simulink model "s_c107m32k_vlbi"  (R2018a)
(part 4 of 201)

      mask help: A 32-bit software-accessible register. Can be divided into bitfields of varying widths and types using the fields in the block mask.
      mask init:
      | swreg_init(gcb)
      settings: AttributesFormatString=2 inputs:uf16.0,uf16.0 = 32 bits
      mask TypeOptions io_dir: To Processor | From Processor
      mask Callback io_dir:
      | mask_enables = get_param(gcb, 'MaskEnables');
      | mask_names = get_param(gcb, 'MaskNames');
      | if strcmp(get_param(gcb, 'io_dir'), 'To Processor'),
      |     mask_enables{ismember(mask_names, 'sample_period')} = 'off';
      | else
      |     mask_enables{ismember(mask_names, 'sample_period')} = 'on';
      | end
      | set_param(gcb, 'MaskEnables', mask_enables);
      mask DialogControl ParameterTabVar0 Prompt: Setup
  tx_metadata : Subsystem  Tag=xps:sw_reg  AncestorBlock=xps_library/Memory/software_register  mask(swreg){io_dir=From Processor, io_delay=0, init_val=0, sample_period=1, names=[porttx board_id], bitwidths=[16 8], bin_pts=0, arith_types=0, sim_port=off, show_format=on}
      mask prompts: io_dir "I/O direction"; io_delay "I/O delay"; init_val "Initial Value"; sample_period "Sample period"; names "Bitfield names [msb...lsb]"; bitwidths "Bitfield widths"; bin_pts "Bitfield binary pts"; arith_types "Bitfield types, ufix=0, fix=1, bool=2"; sim_port "Provide sim input/output?"; show_format "Print format string?"
      mask help: A 32-bit software-accessible register. Can be divided into bitfields of varying widths and types using the fields in the block mask.
      mask init:
      | swreg_init(gcb)
      settings: AttributesFormatString=2 inputs:uf16.0,uf8.0 = 24 bits
      mask TypeOptions io_dir: To Processor | From Processor
      mask Callback io_dir:
      | mask_enables = get_param(gcb, 'MaskEnables');
      | mask_names = get_param(gcb, 'MaskNames');
      | if strcmp(get_param(gcb, 'io_dir'), 'To Processor'),
      |     mask_enables{ismember(mask_names, 'sample_period')} = 'off';
      | else
      |     mask_enables{ismember(mask_names, 'sample_period')} = 'on';
      | end
      | set_param(gcb, 'MaskEnables', mask_enables);
      mask DialogControl ParameterTabVar0 Prompt: Setup
  unpack : Subsystem
  unpack_status : Subsystem  Tag=xps:sw_reg  AncestorBlock=xps_library/Memory/software_register  mask(swreg){io_dir=To Processor, io_delay=0, init_val=0, sample_period=1, names=[magic_err_cnt header_err_cnt pad_err_cnt pkt_len_err_cnt time_err_cnt], bitwidths=6, bin_pts=0, arith_types=0, sim_port=off, show_format=on}
      mask prompts: io_dir "I/O direction"; io_delay "I/O delay"; init_val "Initial Value"; sample_period "Sample period"; names "Bitfield names [msb...lsb]"; bitwidths "Bitfield widths"; bin_pts "Bitfield binary pts"; arith_types "Bitfield types, ufix=0, fix=1, bool=2"; sim_port "Provide sim input/output?"; show_format "Print format string?"
      mask help: A 32-bit software-accessible register. Can be divided into bitfields of varying widths and types using the fields in the block mask.
      mask init:
      | swreg_init(gcb)
      settings: AttributesFormatString=5 outputs:uf6.0,uf6.0,uf6.0,uf6.0,uf6.0 = 30 bits
      mask TypeOptions io_dir: To Processor | From Processor
      mask Callback io_dir:
      | mask_enables = get_param(gcb, 'MaskEnables');
      | mask_names = get_param(gcb, 'MaskNames');
      | if strcmp(get_param(gcb, 'io_dir'), 'To Processor'),
      |     mask_enables{ismember(mask_names, 'sample_period')} = 'off';
      | else
      |     mask_enables{ismember(mask_names, 'sample_period')} = 'on';
      | end
      | set_param(gcb, 'MaskEnables', mask_enables);
      mask DialogControl ParameterTabVar0 Prompt: Setup
  unpack_status1 : Subsystem  Tag=xps:sw_reg  AncestorBlock=xps_library/Memory/software_register  mask(swreg){io_dir=To Processor, io_delay=0, init_val=0, sample_period=1, names=pkt_cnt, bitwidths=32, bin_pts=0, arith_types=0, sim_port=off, show_format=on}
      mask prompts: io_dir "I/O direction"; io_delay "I/O delay"; init_val "Initial Value"; sample_period "Sample period"; names "Bitfield names [msb...lsb]"; bitwidths "Bitfield widths"; bin_pts "Bitfield binary pts"; arith_types "Bitfield types, ufix=0, fix=1, bool=2"; sim_port "Provide sim input/output?"; show_format "Print format string?"
      mask help: A 32-bit software-accessible register. Can be divided into bitfields of varying widths and types using the fields in the block mask.
      mask init:
      | swreg_init(gcb)
      settings: AttributesFormatString=1output:uf32.0 = 32 bits
      mask TypeOptions io_dir: To Processor | From Processor
      mask Callback io_dir:
      | mask_enables = get_param(gcb, 'MaskEnables');
      | mask_names = get_param(gcb, 'MaskNames');
      | if strcmp(get_param(gcb, 'io_dir'), 'To Processor'),
      |     mask_enables{ismember(mask_names, 'sample_period')} = 'off';
      | else
      |     mask_enables{ismember(mask_names, 'sample_period')} = 'on';
      | end
      | set_param(gcb, 'MaskEnables', mask_enables);
      mask DialogControl ParameterTabVar0 Prompt: Setup
  we_delay1 : Subsystem  Tag=cmac_delinked  Commented=on  mask(pipeline){csp_latency=2}
      mask prompts: csp_latency "Latency"
      mask help:
      | An explicitly laid-out delay line to avoid mapping to SRL16s
      | for use in pipelining to help achieve timing closure.
      mask init:
      | pipeline_init(gcb,'latency',csp_latency);
      settings: AttributesFormatString=Latency = %<latency>
      mask Display:
      | port_label('input', 1, 'd');
      | port_label('output', 1, 'q');
      | disp(['Z^-', num2str(csp_latency)]);
  we_delay10 : Subsystem  Tag=cmac_delinked  Commented=on  mask(pipeline){csp_latency=1}
      mask prompts: csp_latency "Latency"
      mask help:
      | An explicitly laid-out delay line to avoid mapping to SRL16s
      | for use in pipelining to help achieve timing closure.
      mask init:
      | pipeline_init(gcb,'latency',csp_latency);
      settings: AttributesFormatString=Latency = %<latency>
      mask Display:
      | port_label('input', 1, 'd');
      | port_label('output', 1, 'q');
      | disp(['Z^-', num2str(csp_latency)]);
  we_delay11 : Subsystem  Tag=cmac_delinked  Commented=on  mask(pipeline){csp_latency=1}
      mask prompts: csp_latency "Latency"
      mask help:
      | An explicitly laid-out delay line to avoid mapping to SRL16s
      | for use in pipelining to help achieve timing closure.
      mask init:
      | pipeline_init(gcb,'latency',csp_latency);
      settings: AttributesFormatString=Latency = %<latency>
      mask Display:
      | port_label('input', 1, 'd');
      | port_label('output', 1, 'q');
      | disp(['Z^-', num2str(csp_latency)]);
  we_delay112 : Subsystem  Tag=cmac_delinked  mask(pipeline){csp_latency=2}
      mask prompts: csp_latency "Latency"
      mask help:
      | An explicitly laid-out delay line to avoid mapping to SRL16s
      | for use in pipelining to help achieve timing closure.
      mask init:
      | pipeline_init(gcb,'latency',csp_latency);
      settings: AttributesFormatString=Latency = %<latency>
      mask Display:
      | port_label('input', 1, 'd');
      | port_label('output', 1, 'q');
      | disp(['Z^-', num2str(csp_latency)]);
  we_delay113 : Subsystem  Tag=cmac_delinked  mask(pipeline){csp_latency=2}
      mask prompts: csp_latency "Latency"
      mask help:
      | An explicitly laid-out delay line to avoid mapping to SRL16s
      | for use in pipelining to help achieve timing closure.
      mask init:
      | pipeline_init(gcb,'latency',csp_latency);
      settings: AttributesFormatString=Latency = %<latency>
      mask Display:
      | port_label('input', 1, 'd');
      | port_label('output', 1, 'q');
      | disp(['Z^-', num2str(csp_latency)]);
  we_delay114 : Subsystem  Tag=cmac_delinked  mask(pipeline){csp_latency=2}
      mask prompts: csp_latency "Latency"
      mask help:
      | An explicitly laid-out delay line to avoid mapping to SRL16s
      | for use in pipelining to help achieve timing closure.
      mask init:
      | pipeline_init(gcb,'latency',csp_latency);
      settings: AttributesFormatString=Latency = %<latency>
      mask Display:
      | port_label('input', 1, 'd');
      | port_label('output', 1, 'q');
      | disp(['Z^-', num2str(csp_latency)]);
  we_delay115 : Subsystem  Tag=cmac_delinked  mask(pipeline){csp_latency=2}
      mask prompts: csp_latency "Latency"
      mask help:
      | An explicitly laid-out delay line to avoid mapping to SRL16s
      | for use in pipelining to help achieve timing closure.
      mask init:
      | pipeline_init(gcb,'latency',csp_latency);
      settings: AttributesFormatString=Latency = %<latency>
      mask Display:
      | port_label('input', 1, 'd');
      | port_label('output', 1, 'q');
      | disp(['Z^-', num2str(csp_latency)]);
  we_delay116 : Subsystem  Tag=cmac_delinked  mask(pipeline){csp_latency=2}
      mask prompts: csp_latency "Latency"
      mask help:
      | An explicitly laid-out delay line to avoid mapping to SRL16s
      | for use in pipelining to help achieve timing closure.
      mask init:
      | pipeline_init(gcb,'latency',csp_latency);
      settings: AttributesFormatString=Latency = %<latency>
      mask Display:
      | port_label('input', 1, 'd');
      | port_label('output', 1, 'q');
      | disp(['Z^-', num2str(csp_latency)]);
  we_delay117 : Subsystem  Tag=cmac_delinked  mask(pipeline){csp_latency=2}
      mask prompts: csp_latency "Latency"
      mask help:
      | An explicitly laid-out delay line to avoid mapping to SRL16s
      | for use in pipelining to help achieve timing closure.
      mask init:
      | pipeline_init(gcb,'latency',csp_latency);
      settings: AttributesFormatString=Latency = %<latency>
      mask Display:
      | port_label('input', 1, 'd');
      | port_label('output', 1, 'q');
      | disp(['Z^-', num2str(csp_latency)]);
  we_delay12 : Subsystem  Tag=cmac_delinked  Commented=on  mask(pipeline){csp_latency=1}
      mask prompts: csp_latency "Latency"
      mask help:
      | An explicitly laid-out delay line to avoid mapping to SRL16s
      | for use in pipelining to help achieve timing closure.
      mask init:
      | pipeline_init(gcb,'latency',csp_latency);
      settings: AttributesFormatString=Latency = %<latency>
      mask Display:
      | port_label('input', 1, 'd');
      | port_label('output', 1, 'q');
      | disp(['Z^-', num2str(csp_latency)]);
  we_delay124 : Subsystem  Tag=cmac_delinked  mask(pipeline){csp_latency=2}
      mask prompts: csp_latency "Latency"
      mask help:
      | An explicitly laid-out delay line to avoid mapping to SRL16s
      | for use in pipelining to help achieve timing closure.
      mask init:
      | pipeline_init(gcb,'latency',csp_latency);
      settings: AttributesFormatString=Latency = %<latency>
      mask Display:
      | port_label('input', 1, 'd');
      | port_label('output', 1, 'q');
      | disp(['Z^-', num2str(csp_latency)]);
  we_delay126 : Subsystem  Tag=cmac_delinked  mask(pipeline){csp_latency=2}
      mask prompts: csp_latency "Latency"
      mask help:
      | An explicitly laid-out delay line to avoid mapping to SRL16s
      | for use in pipelining to help achieve timing closure.
      mask init:
      | pipeline_init(gcb,'latency',csp_latency);
      settings: AttributesFormatString=Latency = %<latency>
      mask Display:
      | port_label('input', 1, 'd');
      | port_label('output', 1, 'q');
      | disp(['Z^-', num2str(csp_latency)]);
  we_delay13 : Subsystem  Tag=cmac_delinked  mask(pipeline){csp_latency=2}
      mask prompts: csp_latency "Latency"
      mask help:
      | An explicitly laid-out delay line to avoid mapping to SRL16s
      | for use in pipelining to help achieve timing closure.
      mask init:
      | pipeline_init(gcb,'latency',csp_latency);
      settings: AttributesFormatString=Latency = %<latency>
      mask Display:
      | port_label('input', 1, 'd');
      | port_label('output', 1, 'q');
      | disp(['Z^-', num2str(csp_latency)]);
  we_delay14 : Subsystem  Tag=cmac_delinked  Commented=on  mask(pipeline){csp_latency=1}
      mask prompts: csp_latency "Latency"
      mask help:
      | An explicitly laid-out delay line to avoid mapping to SRL16s
      | for use in pipelining to help achieve timing closure.
      mask init:
      | pipeline_init(gcb,'latency',csp_latency);
      settings: AttributesFormatString=Latency = %<latency>
      mask Display:
      | port_label('input', 1, 'd');
      | port_label('output', 1, 'q');
      | disp(['Z^-', num2str(csp_latency)]);
  we_delay15 : Subsystem  Tag=cmac_delinked  Commented=on  mask(pipeline){csp_latency=1}
      mask prompts: csp_latency "Latency"
      mask help:
      | An explicitly laid-out delay line to avoid mapping to SRL16s
      | for use in pipelining to help achieve timing closure.
      mask init:
      | pipeline_init(gcb,'latency',csp_latency);
      settings: AttributesFormatString=Latency = %<latency>
      mask Display:
      | port_label('input', 1, 'd');
      | port_label('output', 1, 'q');
      | disp(['Z^-', num2str(csp_latency)]);
  we_delay2 : Subsystem  Tag=cmac_delinked  Commented=on  mask(pipeline){csp_latency=1}
      mask prompts: csp_latency "Latency"
      mask help:
      | An explicitly laid-out delay line to avoid mapping to SRL16s
      | for use in pipelining to help achieve timing closure.
      mask init:
      | pipeline_init(gcb,'latency',csp_latency);
      settings: AttributesFormatString=Latency = %<latency>
      mask Display:
      | port_label('input', 1, 'd');
      | port_label('output', 1, 'q');
      | disp(['Z^-', num2str(csp_latency)]);
  we_delay25 : Subsystem  Tag=cmac_delinked  Commented=on  mask(pipeline){csp_latency=2}
      mask prompts: csp_latency "Latency"
      mask help:
      | An explicitly laid-out delay line to avoid mapping to SRL16s
      | for use in pipelining to help achieve timing closure.
      mask init:
      | pipeline_init(gcb,'latency',csp_latency);
      settings: AttributesFormatString=Latency = %<latency>
      mask Display:
      | port_label('input', 1, 'd');
      | port_label('output', 1, 'q');
      | disp(['Z^-', num2str(csp_latency)]);
  we_delay3 : Subsystem  Tag=cmac_delinked  Commented=on  mask(pipeline){csp_latency=1}
      mask prompts: csp_latency "Latency"
      mask help:
      | An explicitly laid-out delay line to avoid mapping to SRL16s
      | for use in pipelining to help achieve timing closure.
      mask init:
      | pipeline_init(gcb,'latency',csp_latency);
      settings: AttributesFormatString=Latency = %<latency>
      mask Display:
      | port_label('input', 1, 'd');
      | port_label('output', 1, 'q');
      | disp(['Z^-', num2str(csp_latency)]);
  we_delay35 : Subsystem  Tag=cmac_delinked  Commented=on  mask(pipeline){csp_latency=2}
      mask prompts: csp_latency "Latency"
      mask help:
      | An explicitly laid-out delay line to avoid mapping to SRL16s
      | for use in pipelining to help achieve timing closure.
      mask init:
      | pipeline_init(gcb,'latency',csp_latency);
      settings: AttributesFormatString=Latency = %<latency>
      mask Display:
      | port_label('input', 1, 'd');
      | port_label('output', 1, 'q');
      | disp(['Z^-', num2str(csp_latency)]);
  we_delay37 : Subsystem  Tag=cmac_delinked  mask(pipeline){csp_latency=2}
      mask prompts: csp_latency "Latency"
      mask help:
      | An explicitly laid-out delay line to avoid mapping to SRL16s
      | for use in pipelining to help achieve timing closure.
      mask init:
      | pipeline_init(gcb,'latency',csp_latency);
      settings: AttributesFormatString=Latency = %<latency>
      mask Display:
      | port_label('input', 1, 'd');
      | port_label('output', 1, 'q');
      | disp(['Z^-', num2str(csp_latency)]);
  we_delay38 : Subsystem  Tag=cmac_delinked  mask(pipeline){csp_latency=2}
      mask prompts: csp_latency "Latency"
      mask help:
      | An explicitly laid-out delay line to avoid mapping to SRL16s
      | for use in pipelining to help achieve timing closure.
      mask init:
      | pipeline_init(gcb,'latency',csp_latency);
      settings: AttributesFormatString=Latency = %<latency>
      mask Display:
      | port_label('input', 1, 'd');
      | port_label('output', 1, 'q');
      | disp(['Z^-', num2str(csp_latency)]);
  we_delay39 : Subsystem  Tag=cmac_delinked  mask(pipeline){csp_latency=2}
      mask prompts: csp_latency "Latency"
      mask help:
      | An explicitly laid-out delay line to avoid mapping to SRL16s
      | for use in pipelining to help achieve timing closure.
      mask init:
      | pipeline_init(gcb,'latency',csp_latency);
      settings: AttributesFormatString=Latency = %<latency>
      mask Display:
      | port_label('input', 1, 'd');
      | port_label('output', 1, 'q');
      | disp(['Z^-', num2str(csp_latency)]);
  we_delay4 : Subsystem  Tag=cmac_delinked  Commented=on  mask(pipeline){csp_latency=1}
      mask prompts: csp_latency "Latency"
      mask help:
      | An explicitly laid-out delay line to avoid mapping to SRL16s
      | for use in pipelining to help achieve timing closure.
      mask init:
      | pipeline_init(gcb,'latency',csp_latency);
      settings: AttributesFormatString=Latency = %<latency>
      mask Display:
      | port_label('input', 1, 'd');
      | port_label('output', 1, 'q');
      | disp(['Z^-', num2str(csp_latency)]);
  we_delay41 : Subsystem  Tag=cmac_delinked  mask(pipeline){csp_latency=2}
      mask prompts: csp_latency "Latency"
      mask help:
      | An explicitly laid-out delay line to avoid mapping to SRL16s
      | for use in pipelining to help achieve timing closure.
      mask init:
      | pipeline_init(gcb,'latency',csp_latency);
      settings: AttributesFormatString=Latency = %<latency>
      mask Display:
      | port_label('input', 1, 'd');
      | port_label('output', 1, 'q');
      | disp(['Z^-', num2str(csp_latency)]);
  we_delay47 : Subsystem  Tag=cmac_delinked  mask(pipeline){csp_latency=2}
      mask prompts: csp_latency "Latency"
      mask help:
      | An explicitly laid-out delay line to avoid mapping to SRL16s
      | for use in pipelining to help achieve timing closure.
      mask init:
      | pipeline_init(gcb,'latency',csp_latency);
      settings: AttributesFormatString=Latency = %<latency>
      mask Display:
      | port_label('input', 1, 'd');
      | port_label('output', 1, 'q');
      | disp(['Z^-', num2str(csp_latency)]);
  we_delay48 : Subsystem  Tag=cmac_delinked  mask(pipeline){csp_latency=2}
      mask prompts: csp_latency "Latency"
      mask help:
      | An explicitly laid-out delay line to avoid mapping to SRL16s
      | for use in pipelining to help achieve timing closure.
      mask init:
      | pipeline_init(gcb,'latency',csp_latency);
      settings: AttributesFormatString=Latency = %<latency>
      mask Display:
      | port_label('input', 1, 'd');
      | port_label('output', 1, 'q');
      | disp(['Z^-', num2str(csp_latency)]);
  we_delay49 : Subsystem  Tag=cmac_delinked  mask(pipeline){csp_latency=2}
      mask prompts: csp_latency "Latency"
      mask help:
      | An explicitly laid-out delay line to avoid mapping to SRL16s
      | for use in pipelining to help achieve timing closure.
      mask init:
      | pipeline_init(gcb,'latency',csp_latency);
      settings: AttributesFormatString=Latency = %<latency>
      mask Display:
      | port_label('input', 1, 'd');
      | port_label('output', 1, 'q');
      | disp(['Z^-', num2str(csp_latency)]);
  we_delay5 : Subsystem  Tag=cmac_delinked  Commented=on  mask(pipeline){csp_latency=1}
      mask prompts: csp_latency "Latency"
      mask help:
      | An explicitly laid-out delay line to avoid mapping to SRL16s
      | for use in pipelining to help achieve timing closure.
      mask init:
      | pipeline_init(gcb,'latency',csp_latency);
      settings: AttributesFormatString=Latency = %<latency>
      mask Display:
      | port_label('input', 1, 'd');
      | port_label('output', 1, 'q');
      | disp(['Z^-', num2str(csp_latency)]);
  we_delay50 : Subsystem  Tag=cmac_delinked  mask(pipeline){csp_latency=2}
      mask prompts: csp_latency "Latency"
      mask help:
      | An explicitly laid-out delay line to avoid mapping to SRL16s
      | for use in pipelining to help achieve timing closure.
      mask init:
      | pipeline_init(gcb,'latency',csp_latency);
      settings: AttributesFormatString=Latency = %<latency>
      mask Display:
      | port_label('input', 1, 'd');
      | port_label('output', 1, 'q');
      | disp(['Z^-', num2str(csp_latency)]);
  we_delay54 : Subsystem  Tag=cmac_delinked  Commented=on  mask(pipeline){csp_latency=2}
      mask prompts: csp_latency "Latency"
      mask help:
      | An explicitly laid-out delay line to avoid mapping to SRL16s
      | for use in pipelining to help achieve timing closure.
      mask init:
      | pipeline_init(gcb,'latency',csp_latency);
      settings: AttributesFormatString=Latency = %<latency>
      mask Display:
      | port_label('input', 1, 'd');
      | port_label('output', 1, 'q');
      | disp(['Z^-', num2str(csp_latency)]);
  we_delay55 : Subsystem  Tag=cmac_delinked  Commented=on  mask(pipeline){csp_latency=2}
      mask prompts: csp_latency "Latency"
      mask help:
      | An explicitly laid-out delay line to avoid mapping to SRL16s
      | for use in pipelining to help achieve timing closure.
      mask init:
      | pipeline_init(gcb,'latency',csp_latency);
      settings: AttributesFormatString=Latency = %<latency>
      mask Display:
      | port_label('input', 1, 'd');
      | port_label('output', 1, 'q');
      | disp(['Z^-', num2str(csp_latency)]);
  we_delay56 : Subsystem  Tag=cmac_delinked  Commented=on  mask(pipeline){csp_latency=2}
      mask prompts: csp_latency "Latency"
      mask help:
      | An explicitly laid-out delay line to avoid mapping to SRL16s
      | for use in pipelining to help achieve timing closure.
      mask init:
      | pipeline_init(gcb,'latency',csp_latency);
      settings: AttributesFormatString=Latency = %<latency>
      mask Display:
      | port_label('input', 1, 'd');
      | port_label('output', 1, 'q');
      | disp(['Z^-', num2str(csp_latency)]);
  we_delay57 : Subsystem  Tag=cmac_delinked  Commented=on  mask(pipeline){csp_latency=2}
      mask prompts: csp_latency "Latency"
      mask help:
      | An explicitly laid-out delay line to avoid mapping to SRL16s
      | for use in pipelining to help achieve timing closure.
      mask init:
      | pipeline_init(gcb,'latency',csp_latency);
      settings: AttributesFormatString=Latency = %<latency>
      mask Display:
      | port_label('input', 1, 'd');
      | port_label('output', 1, 'q');
      | disp(['Z^-', num2str(csp_latency)]);
  we_delay6 : Subsystem  Tag=cmac_delinked  Commented=on  mask(pipeline){csp_latency=1}
      mask prompts: csp_latency "Latency"
      mask help:
      | An explicitly laid-out delay line to avoid mapping to SRL16s
      | for use in pipelining to help achieve timing closure.
      mask init:
      | pipeline_init(gcb,'latency',csp_latency);
      settings: AttributesFormatString=Latency = %<latency>
      mask Display:
      | port_label('input', 1, 'd');
      | port_label('output', 1, 'q');
      | disp(['Z^-', num2str(csp_latency)]);
  we_delay68 : Subsystem  Tag=cmac_delinked  Commented=on  mask(pipeline){csp_latency=2}
      mask prompts: csp_latency "Latency"
      mask help:
      | An explicitly laid-out delay line to avoid mapping to SRL16s
      | for use in pipelining to help achieve timing closure.
      mask init:
      | pipeline_init(gcb,'latency',csp_latency);
      settings: AttributesFormatString=Latency = %<latency>
      mask Display:
      | port_label('input', 1, 'd');
      | port_label('output', 1, 'q');
      | disp(['Z^-', num2str(csp_latency)]);
  we_delay69 : Subsystem  Tag=cmac_delinked  Commented=on  mask(pipeline){csp_latency=2}
      mask prompts: csp_latency "Latency"
      mask help:
      | An explicitly laid-out delay line to avoid mapping to SRL16s
      | for use in pipelining to help achieve timing closure.
      mask init:
      | pipeline_init(gcb,'latency',csp_latency);
      settings: AttributesFormatString=Latency = %<latency>
      mask Display:
      | port_label('input', 1, 'd');
      | port_label('output', 1, 'q');
      | disp(['Z^-', num2str(csp_latency)]);
  we_delay7 : Subsystem  Tag=cmac_delinked  Commented=on  mask(pipeline){csp_latency=1}
      mask prompts: csp_latency "Latency"
      mask help:
      | An explicitly laid-out delay line to avoid mapping to SRL16s
      | for use in pipelining to help achieve timing closure.
      mask init:
      | pipeline_init(gcb,'latency',csp_latency);
      settings: AttributesFormatString=Latency = %<latency>
      mask Display:
      | port_label('input', 1, 'd');
      | port_label('output', 1, 'q');
      | disp(['Z^-', num2str(csp_latency)]);
  we_delay77 : Subsystem  Tag=cmac_delinked  mask(pipeline){csp_latency=2}
      mask prompts: csp_latency "Latency"
      mask help:
      | An explicitly laid-out delay line to avoid mapping to SRL16s
      | for use in pipelining to help achieve timing closure.
      mask init:
      | pipeline_init(gcb,'latency',csp_latency);
      settings: AttributesFormatString=Latency = %<latency>
      mask Display:
      | port_label('input', 1, 'd');
      | port_label('output', 1, 'q');
      | disp(['Z^-', num2str(csp_latency)]);
  we_delay78 : Subsystem  Tag=cmac_delinked  mask(pipeline){csp_latency=2}
      mask prompts: csp_latency "Latency"
      mask help:
      | An explicitly laid-out delay line to avoid mapping to SRL16s
      | for use in pipelining to help achieve timing closure.
      mask init:
      | pipeline_init(gcb,'latency',csp_latency);
      settings: AttributesFormatString=Latency = %<latency>
      mask Display:
      | port_label('input', 1, 'd');
      | port_label('output', 1, 'q');
      | disp(['Z^-', num2str(csp_latency)]);
  we_delay79 : Subsystem  Tag=cmac_delinked  Commented=on  mask(pipeline){csp_latency=2}
      mask prompts: csp_latency "Latency"
      mask help:
      | An explicitly laid-out delay line to avoid mapping to SRL16s
      | for use in pipelining to help achieve timing closure.
      mask init:
      | pipeline_init(gcb,'latency',csp_latency);
      settings: AttributesFormatString=Latency = %<latency>
      mask Display:
      | port_label('input', 1, 'd');
      | port_label('output', 1, 'q');
      | disp(['Z^-', num2str(csp_latency)]);
  we_delay8 : Subsystem  Tag=cmac_delinked  Commented=on  mask(pipeline){csp_latency=1}
      mask prompts: csp_latency "Latency"
      mask help:
      | An explicitly laid-out delay line to avoid mapping to SRL16s
      | for use in pipelining to help achieve timing closure.
      mask init:
      | pipeline_init(gcb,'latency',csp_latency);
      settings: AttributesFormatString=Latency = %<latency>
      mask Display:
      | port_label('input', 1, 'd');
      | port_label('output', 1, 'q');
      | disp(['Z^-', num2str(csp_latency)]);
  we_delay80 : Subsystem  Tag=cmac_delinked  Commented=on  mask(pipeline){csp_latency=2}
      mask prompts: csp_latency "Latency"
      mask help:
      | An explicitly laid-out delay line to avoid mapping to SRL16s
      | for use in pipelining to help achieve timing closure.
      mask init:
      | pipeline_init(gcb,'latency',csp_latency);
      settings: AttributesFormatString=Latency = %<latency>
      mask Display:
      | port_label('input', 1, 'd');
      | port_label('output', 1, 'q');
      | disp(['Z^-', num2str(csp_latency)]);
  we_delay81 : Subsystem  Tag=cmac_delinked  Commented=on  mask(pipeline){csp_latency=2}
      mask prompts: csp_latency "Latency"
      mask help:
      | An explicitly laid-out delay line to avoid mapping to SRL16s
      | for use in pipelining to help achieve timing closure.
      mask init:
      | pipeline_init(gcb,'latency',csp_latency);
      settings: AttributesFormatString=Latency = %<latency>
      mask Display:
      | port_label('input', 1, 'd');
      | port_label('output', 1, 'q');
      | disp(['Z^-', num2str(csp_latency)]);
  we_delay9 : Subsystem  Tag=cmac_delinked  Commented=on  mask(pipeline){csp_latency=1}
      mask prompts: csp_latency "Latency"
      mask help:
      | An explicitly laid-out delay line to avoid mapping to SRL16s
      | for use in pipelining to help achieve timing closure.
      mask init:
      | pipeline_init(gcb,'latency',csp_latency);
      settings: AttributesFormatString=Latency = %<latency>
      mask Display:
      | port_label('input', 1, 'd');
      | port_label('output', 1, 'q');
      | disp(['Z^-', num2str(csp_latency)]);
  x_setup : Subsystem  Tag=xps:sw_reg  AncestorBlock=xps_library/Memory/software_register  mask(swreg){io_dir=From Processor, io_delay=0, init_val=0, sample_period=1, names=[f_per_x ip_per_x num_x snap_arm pktstart_mux pack_mux pktoffset_sel], bitwidths=[15 4 9 1 1 1 1], bin_pts=[0 2 0 0 0 0 0], arith_types=[0 0 0 2 0 2 0], sim_port=off, show_format=on}
      mask prompts: io_dir "I/O direction"; io_delay "I/O delay"; init_val "Initial Value"; sample_period "Sample period"; names "Bitfield names [msb...lsb]"; bitwidths "Bitfield widths"; bin_pts "Bitfield binary pts"; arith_types "Bitfield types, ufix=0, fix=1, bool=2"; sim_port "Provide sim input/output?"; show_format "Print format string?"
      mask help: A 32-bit software-accessible register. Can be divided into bitfields of varying widths and types using the fields in the block mask.
      mask init:
      | swreg_init(gcb)
      settings: AttributesFormatString=7 inputs:uf15.0,uf4.2,uf9.0,b,uf1.0,b,uf1.0 = 32 bits
      mask TypeOptions io_dir: To Processor | From Processor
      mask Callback io_dir:
      | mask_enables = get_param(gcb, 'MaskEnables');
      | mask_names = get_param(gcb, 'MaskNames');
      | if strcmp(get_param(gcb, 'io_dir'), 'To Processor'),
      |     mask_enables{ismember(mask_names, 'sample_period')} = 'off';
      | else
      |     mask_enables{ismember(mask_names, 'sample_period')} = 'on';
      | end
      | set_param(gcb, 'MaskEnables', mask_enables);
      mask DialogControl ParameterTabVar0 Prompt: Setup
  xeng_match : Subsystem  Tag=xps:sw_reg  AncestorBlock=xps_library/Memory/software_register  mask(swreg){io_dir=From Processor, io_delay=0, init_val=0, sample_period=1, names=[val], bitwidths=[3], bin_pts=0, arith_types=0, sim_port=on, show_format=on}
      mask prompts: io_dir "I/O direction"; io_delay "I/O delay"; init_val "Initial Value"; sample_period "Sample period"; names "Bitfield names [msb...lsb]"; bitwidths "Bitfield widths"; bin_pts "Bitfield binary pts"; arith_types "Bitfield types, ufix=0, fix=1, bool=2"; sim_port "Provide sim input/output?"; show_format "Print format string?"
      mask help: A 32-bit software-accessible register. Can be divided into bitfields of varying widths and types using the fields in the block mask.
      mask init:
      | swreg_init(gcb)
      settings: AttributesFormatString=1input:uf3.0 = 3 bits
      mask TypeOptions io_dir: To Processor | From Processor
      mask Callback io_dir:
      | mask_enables = get_param(gcb, 'MaskEnables');
      | mask_names = get_param(gcb, 'MaskNames');
      | if strcmp(get_param(gcb, 'io_dir'), 'To Processor'),
      |     mask_enables{ismember(mask_names, 'sample_period')} = 'off';
      | else
      |     mask_enables{ismember(mask_names, 'sample_period')} = 'on';
      | end
      | set_param(gcb, 'MaskEnables', mask_enables);
      mask DialogControl ParameterTabVar0 Prompt: Setup
  xsg_core_config : xps_library/Platforms/SKARAB  Tag=xps:xsg  hw_sys=SKARAB:xc7vx690t  clk_src=sys_clk  clk_rate=238  sample_period=1  synthesis_tool=XST
      settings: SourceProductName=CASPER XPS Blockset
  tag scope: cnt_rst=global, ct_board_hmc_offset=global, ct_chans_per_board=global, ct_chans_per_x=global, ct_chans_per_x_recip=global, ct_fake_data_error=global, ct_freq_gen_offset=global, ct_num_x_boards=global, ct_num_x_boards_recip=global, ct_num_xeng=global, ct_num_xeng_recip=global, ct_rst_err_latch=global, ct_tag_insert_sel=global, ct_tvg_en2=global, ct_tvg_en=global, ct_x_per_board=global, ct_x_per_board_recip=global, ddc_bypass=global, fd_bypass=global, force_gbe_txen=global, local_time_capture=global, local_time_src=global, obuf_read_gap=global, pfb_bypass=global, pktoffset_sel=global, pktstart_sel=global, q_bypass=global, reo_time_change=global, snap_reord_mux_we_sel=global, snap_stop_mux_sel=global, sync80=global, sys_rst=global, tg_dds_time_out=global, tg_rd_time_out=global, time80=global, time80_48=global, ts_tvg_en=global, tvgtone_level0=global, tvgtone_level1=global, tvgtone_p0=global, tvgtone_p1=global, up_timestep_error=global, valid80=global
  wires:
  Counter2/1 -> pipeline29/1(d)
  Constant26/1 -> eq1/2(data_in)
  Constant11/1 -> eq1/3(we)
  Delay53/1 -> quant1/1(sync_in)
  Delay34/1 -> quant1/2(din)
  eq1/1(data_out) -> quant1/4(coeffs)
  Delay50/1 -> quant1/3(en)
  Counter4/1 -> pipeline27/1(d)
  Constant24/1 -> eq0/2(data_in)
  Constant25/1 -> eq0/3(we)
  Delay51/1 -> quant0/1(sync_in)
  Delay2/1 -> quant0/2(din)
  Delay52/1 -> quant0/3(en)
  eq0/1(data_out) -> quant0/4(coeffs)
  quant1/1(sync_out) -> Terminator19/1
  quant1/3(dvalid) -> Terminator21/1
  pipeline27/1(q) -> eq0/1(addr)
  pipeline29/1(q) -> eq1/1(addr)
  pipeline41/1(q) -> Counter4/2
  pipeline42/1(q) -> Counter4/1
  pipeline45/1(q) -> Counter2/2
  pipeline48/1(q) -> Counter2/1
  [delay_sync] -> [pfbin_sync]
  [delay_dv] -> [pfbin_dv]
  [delay_d0] -> [pfbin_d0]
  [delay_d1] -> [pfbin_d1]
  [q_sync] -> generate_pkt_sync1/1(sync)
  Concat4/1 -> generate_pkt_sync1/3(data)
  [q_d64_0] -> Concat4/1
  [q_d64_1] -> Concat4/2
  bus_expand5/1(msb_out2) -> quant_snap_filter0/3(data_in)
  [q_dv] -> generate_pkt_sync1/2(valid)
  generate_pkt_sync1/3(out_data) -> pipeline65/1(d)
  generate_pkt_sync1/2(out_valid) -> pipeline79/1(d), pipeline58/1(d)
  generate_pkt_sync1/4(packet_sync) -> pipeline80/1(d), pipeline64/1(d)
  pipeline65/1(q) -> bus_expand5/1(bus_in)
  bus_expand4/1(msb_out8) -> snap_quant1/1(in_real0)
  bus_expand4/2(out7) -> snap_quant1/2(in_imag0)
  bus_expand4/3(out6) -> snap_quant1/3(in_real1)
  bus_expand4/4(out5) -> snap_quant1/4(in_imag1)
  bus_expand4/5(out4) -> snap_quant1/5(in_real2)
  bus_expand4/6(out3) -> snap_quant1/6(in_imag2)
  bus_expand4/7(out2) -> snap_quant1/7(in_real3)
  bus_expand4/8(lsb_out1) -> snap_quant1/8(in_imag3)
  quant_snap_filter0/2(data_out) -> bus_expand3/1(bus_in)
  quant_snap_filter1/2(data_out) -> bus_expand4/1(bus_in)
  bus_expand5/2(lsb_out1) -> quant_snap_filter1/3(data_in)
  quant_snap_filter1/3(packet_sync_out) -> snap_quant1/10(trig)
  quant_snap_filter1/1(data_valid_out) -> snap_quant1/9(we)
  generate_pkt_sync1/1(out_sync) -> [generate_pkt_sync_out]
  [generate_pkt_sync_out] -> quant_snap_filter0/1(sync_in)
  [generate_pkt_sync_out] -> quant_snap_filter1/1(sync_in)
  pipeline79/1(q) -> [gp_dv0]
  [gp_dv0] -> quant_snap_filter0/2(data_valid_in)
  pipeline80/1(q) -> [gp_pktsync0]
  [gp_pktsync0] -> quant_snap_filter0/4(packet_sync_in)
  pipeline58/1(q) -> [gp_dv1]
  pipeline64/1(q) -> [gp_pktsync1]
  [gp_dv1] -> quant_snap_filter1/2(data_valid_in)
  [gp_pktsync1] -> quant_snap_filter1/4(packet_sync_in)
  [quant_snap_single_channel] -> quant_snap_filter0/5(single_channel_enable)
  [quant_snap_channel_select] -> quant_snap_filter0/6(channel_select)
  [quant_snap_single_channel] -> quant_snap_filter1/5(single_channel_enable)
  [quant_snap_channel_select] -> quant_snap_filter1/6(channel_select)
  Slice3/1 -> [quant_snap_channel_select]
  DDC/1(ddc_sync) -> [ddc_sync]
  DDC/2(ddc_pol0) -> [ddc_pol0]
  DDC/3(ddc_pol1) -> [ddc_pol1]
  DDC/4(ddc_dv) -> [ddc_dvalid]
  Gateway Out65/1 -> To Workspace69/1
  [ddc_dvalid] -> Gateway Out65/1
  Gateway Out4/1 -> To Workspace1/1
  [ddc_pol1] -> Gateway Out4/1
  Gateway Out2/1 -> To Workspace2/1
  [ddc_pol0] -> Gateway Out2/1
  [ddc_sync] -> Gateway Out1/1
  Gateway Out1/1 -> To Workspace3/1
  From270/1 -> pipeline145/1(d)
  From271/1 -> pipeline146/1(d)
  From272/1 -> pipeline144/1(d)
  From273/1 -> pipeline142/1(d)
  [ddc_sync_in] -> DDC/1(sync)
  [ddc_pol1_in] -> DDC/5(pol1_data)
  [ddc_dv_in] -> DDC/2(dvalid)
  [ddc_pol0_in] -> DDC/3(pol0_data)
  From269/1 -> pipeline141/1(d)
  From268/1 -> pipeline140/1(d)
  [clr_status] -> Subsystem15/1(rst)
  Subsystem15/1(out0) -> quant_status/1(out_pol0_or_cnt)
  Relational/1 -> Subsystem15/2(in0)
  Constant59/1 -> Relational/2
  [q_of0] -> Relational/1
  Relational3/1 -> Subsystem15/3(in1)
  [q_of1] -> Relational3/1
  Constant58/1 -> Relational3/2
  Subsystem15/2(out1) -> quant_status/2(out_pol1_or_cnt)
  tl_fd0/1(value) -> fd_nb0/4(delay_value)
  [clr_status] -> tl_fd0/1(cnt_rst), tl_fd1/1(cnt_rst)
  fd_nb1/1(sync_out) -> Terminator24/1
  fd_nb1/3(dvalid) -> Terminator25/1
  [ld_val0] -> tl_fd0/3(load_value)
  bus_expand16/1(msb_out2) -> tl_fd0/5(din)
  bus_expand16/2(lsb_out1) -> tl_fd1/5(din)
  time_gen_nb/3(rd_val_out) -> tl_fd0/2(current_time), tl_fd1/2(current_time), [pfb_time]
  tl_fd0/7(misco) -> Terminator3/1
  tl_fd0/6(time) -> [fdfs_time]
  tl_fd1/6(time) -> Terminator17/1
  tl_fd1/7(misco) -> Terminator20/1
  time_gen_nb/1(rd_sync_out) -> [tg_pfb_sync]
  time_gen_nb/2(rd_dvalid) -> [tg_pfb_dv]
  time_gen_nb/4(rd_misc_out) -> bus_expand16/1(bus_in)
  [sync80] -> pipeline207/1(d)
  [valid80] -> pipeline208/1(d)
  Concat1/1 -> time_gen_nb/6(rd_misc_in)
  pipeline207/1(q) -> time_gen_nb/1(wr_sync_in)
  pipeline208/1(q) -> time_gen_nb/2(wr_en)
  pipeline210/1(q) -> time_gen_nb/4(rd_sync_in)
  pipeline212/1(q) -> time_gen_nb/5(rd_en)
  pipeline228/1(q) -> Concat1/1
  pipeline231/1(q) -> Concat1/2
  tl_fd0/3(sync_out) -> [tlfd_sync], fd_nb0/1(sync_in)
  tl_fd0/4(dout) -> [tlfd_d0], fd_nb0/2(din)
  tl_fd0/5(dvalid) -> [tlfd_dv], fd_nb0/3(en)
  tl_fd0/2(enable) -> fd_nb0/5(load_value)
  [osc_freq] -> [tlfd_osc], fd_nb0/6(mix_freq), fd_nb1/6(mix_freq)
  Constant4/1 -> gbe0/8(rx_overrun_ack)
  Constant19/1 -> gbe0/7(rx_ack)
  [gbe_rst] -> pipeline99/1(d)
  sync_gen/2(dout) -> bus_expand6/1(bus_in)
  sync_gen/3(dvalid) -> impulse_gen1/6(en), impulse_gen0/6(en)
  impulse_gen0/4(misco) -> [time80], [time80_48]
  impulse_gen0/3(dvalid) -> [valid80]
  impulse_gen0/1(sync_out) -> [sync80]
  impulse_gen0/2(dout) -> [d80_adc0]
  [tvg_adc0_en] -> impulse_gen0/1(tvg_en)
  impulse_gen1/1(sync_out) -> Terminator6/1
  impulse_gen1/2(dout) -> [d80_adc1]
  impulse_gen1/3(dvalid) -> Terminator8/1
  impulse_gen1/4(misco) -> [dig_flags]
  [tvg_adc1_en] -> impulse_gen1/1(tvg_en)
  impulse0/1(in_offset) -> Slice7/1
  impulse0/2(in_amplitude) -> impulse_gen0/3(impulse_amplitude)
  impulse1/1(in_offset) -> Slice8/1
  impulse1/2(in_amplitude) -> impulse_gen1/3(impulse_amplitude)
  sync_gen/1(sync) -> impulse_gen0/4(sync_in), impulse_gen1/4(sync_in)
  bus_expand6/1(msb_out2) -> impulse_gen0/5(din)
  bus_expand6/2(lsb_out1) -> impulse_gen1/5(din)
  sync_gen/5(misco) -> impulse_gen1/7(misci)
  sync_gen/4(time_out) -> impulse_gen0/7(misci)
  [unpack_timestamp] -> sync_gen/1(time_in)
  [sys_relock] -> sync_gen/5(relock)
  [unpack_dv] -> sync_gen/2(en)
  [unpack_d160] -> sync_gen/3(din)
  Slice7/1 -> impulse_gen0/2(impulse_offset)
  Slice8/1 -> impulse_gen1/2(impulse_offset)
  [gbe_cnt_rst] -> pipeline31/1(d)
  pipeline31/1(q) -> gbe0/9(debug_rst)
  gbe0/13(rx_dest_ip) -> pipeline115/1(d)
  gbe0/14(rx_dest_port) -> pipeline116/1(d)
  [rx_dest_ip] -> pipeline/1(d)
  pipeline/1(q) -> rx_dest_ip/1(out_reg)
  gbe0/1(led_up) -> pipeline100/1(d)
  [forty_gbe_led_up] -> pipeline19/1(d)
  gbe0/2(led_rx) -> pipeline101/1(d)
  [forty_gbe_led_rx] -> pipeline20/1(d)
  gbe0/3(led_tx) -> pipeline102/1(d)
  [forty_gbe_led_tx] -> pipeline51/1(d)
  gbe0/4(tx_afull) -> pipeline103/1(d)
  gbe0/5(tx_overflow) -> pipeline104/1(d)
  gbe0/12(rx_overrun) -> pipeline114/1(d)
  pipeline19/1(q) -> gbe_status/1(out_led_up)
  pipeline20/1(q) -> gbe_status/2(out_led_rx)
  pipeline51/1(q) -> gbe_status/3(out_led_tx)
  gbe0/8(rx_source_ip) -> pipeline110/1(d)
  gbe0/9(rx_source_port) -> pipeline111/1(d)
  gbe0/6(rx_data) -> pipeline108/1(d)
  gbe0/10(rx_end_of_frame) -> pipeline112/1(d)
  gbe0/11(rx_bad_frame) -> pipeline113/1(d)
  [s256_d] -> pipeline98/1(d)
  [s256_ip] -> pipeline97/1(d)
  [s256_port] -> pipeline96/1(d)
  Logical3/1 -> gbe0/6(tx_end_of_frame)
  [s256_v] -> Logical1/2
  [s256_eof] -> Logical3/2
  Delay1/1 -> Logical1/1, Logical3/1
  [s256_eof] -> Delay1/2
  pipeline96/1(q) -> gbe0/5(tx_dest_port)
  pipeline97/1(q) -> gbe0/4(tx_dest_ip)
  pipeline98/1(q) -> gbe0/2(tx_data)
  pipeline99/1(q) -> gbe0/1(rst)
  Logical5/1 -> Delay1/1
  pipeline100/1(q) -> [forty_gbe_led_up]
  pipeline101/1(q) -> [forty_gbe_led_rx]
  pipeline102/1(q) -> [forty_gbe_led_tx]
  pipeline103/1(q) -> [forty_gbe_tx_full]
  pipeline104/1(q) -> [forty_gbe_tx_of]
  pipeline108/1(q) -> [forty_gbe_rx_data]
  pipeline110/1(q) -> [forty_gbe_rx_src_ip]
  pipeline111/1(q) -> [forty_gbe_rx_src_port]
  pipeline112/1(q) -> [forty_gbe_rx_eof]
  pipeline113/1(q) -> [forty_gbe_rx_bad]
  pipeline114/1(q) -> [forty_gbe_rx_overrun]
  pipeline115/1(q) -> [rx_dest_ip]
  pipeline116/1(q) -> [rx_dest_port]
  [forty_gbe_rx_data] -> unpack/1(d256)
  [forty_gbe_rx_valid] -> unpack/2(dv256)
  [forty_gbe_rx_eof] -> unpack/3(eof256)
  Constant1/1 -> sync_gen/4(misci)
  Logical1/1 -> gbe0/3(tx_valid)
  Subsystem7/1(per_sec) -> reorder_status1/1(out_dv_per_sec)
  [upg_reo_time] -> Subsystem1/3(time)
  [upg_reo_recv] -> Subsystem1/4(recv)
  [upg_reo_dv] -> Subsystem7/1(dv), Subsystem1/2(dv)
  [cnt_rst] -> Subsystem1/1(rst)
  Subsystem1/7(time_change) -> [reo_time_change]
  Logical6/1 -> Subsystem1/7(overflow_err)
  [upg_of80_p1] -> Logical6/2
  [upg_of80_p0] -> Logical6/1
  Subsystem1/8(timestep_err) -> [up_timestep_error]
  [upg_reo_disc] -> Subsystem1/5(discard_err)
  [upg_reo_relock] -> Subsystem1/6(relock_err)
  Subsystem1/1(timestep_err_cnt) -> reorder_status/1(out_timestep_err_cnt)
  Subsystem1/2(recv_err_cnt) -> reorder_status/2(out_receive_err_cnt)
  Subsystem1/3(discard_err_cnt) -> reorder_status/3(out_discard_cnt)
  Subsystem1/4(relock_err_cnt) -> reorder_status/4(out_relock_err_cnt)
  Subsystem1/5(overflow_err_cnt) -> reorder_status/5(out_overflow_err_cnt)
  Subsystem1/6(dv_cnt) -> reorder_status/6(out_dv_cnt)
  gbe0/7(rx_valid) -> pipeline62/1(d)
  pipeline62/1(q) -> [forty_gbe_rx_valid]
  [gbe_txen] -> Logical5/2
  [force_gbe_txen] -> Logical7/2
  Logical7/1 -> Logical5/1
  [upg_sperr_magic] -> Subsystem33/2(in0)
  [upg_sperr_len] -> Subsystem33/5(in3)
  [upg_sperr_hdr] -> Subsystem33/3(in1)
  [upg_sperr_pad] -> Subsystem33/4(in2)
  Subsystem33/5(out4) -> unpack_status/5(out_time_err_cnt)
  [upg_sperr_time] -> Subsystem33/6(in4)
  Subsystem33/4(out3) -> unpack_status/4(out_pkt_len_err_cnt)
  Subsystem33/3(out2) -> unpack_status/3(out_pad_err_cnt)
  Subsystem33/2(out1) -> unpack_status/2(out_header_err_cnt)
  Subsystem33/1(out0) -> unpack_status/1(out_magic_err_cnt)
  [cnt_rst] -> Subsystem4/1(rst), Subsystem33/1(rst)
  Logical4/1 -> Subsystem4/2(in0)
  Subsystem4/1(out0) -> unpack_status1/1(out_pkt_cnt)
  [upg_sp_dv] -> Logical4/2
  [upg_sp_eof] -> Logical4/1
  Slice17/1 -> local_time_lsw/1(out_timestamp_lsw)
  Slice15/1 -> Convert1/1
  [local_time_capture] -> Delay31/1
  unpack/5(spead_timestamp) -> [spead_timestamp]
  pipeline16/1(q) -> Slice17/1, Slice15/1
  [local_time_src] -> Mux/1
  [time80_48] -> Delay9/1
  [valid80] -> Delay9/2
  [pfb_time] -> Delay10/1
  [pfb_dv] -> Delay10/2
  [flag_dvalid] -> Delay11/2
  [pack_sync_time] -> Delay11/1
  Convert1/1 -> local_time_msw/1(out_timestamp_msw)
  AddSub/1 -> Relational4/2, Relational2/1, time_difference/1(out_time_difference), pipeline204/1(d)
  Logical/1 -> [time_diff_error]
  time_check/1(in_max_difference) -> Relational2/2
  [time_diff_check_en] -> Logical/2
  sync_gen/6(waiting) -> [sync_armed]
  Delay31/1 -> Register3/2, Register2/2, Register4/2, Register1/2
  Delay10/1 -> Register2/1
  [spead_timestamp] -> Register4/1
  Register4/1 -> Mux/2
  Register1/1 -> Mux/3
  Register2/1 -> Mux/4
  Register3/1 -> Mux/5
  Mux/1 -> pipeline16/1(d)
  unpack/4(recvd) -> ts_tvg/6(recvd_in)
  unpack/1(d160) -> ts_tvg/3(data_in)
  unpack/2(dv) -> ts_tvg/4(dv_in)
  unpack/3(time) -> ts_tvg/5(time_in)
  pipeline11/1(q) -> [unpack_d160]
  pipeline12/1(q) -> [unpack_dv]
  pipeline15/1(q) -> [unpack_timestamp]
  ts_tvg/1(d160) -> pipeline11/1(d)
  ts_tvg/2(dv) -> pipeline12/1(d)
  ts_tvg/3(time) -> pipeline15/1(d)
  ts_tvg/4(recvd) -> Terminator9/1
  [ts_tvg_en] -> ts_tvg/1(tvg_en)
  [pipeline_stall] -> ts_tvg/2(stall_pipeline)
  [board_in_fault] -> Inverter/1
  Inverter/1 -> Logical7/1
  From101/1 -> Relational1/1, Delay32/1
  From117/1 -> Delay35/1
  From105/1 -> Delay32/2, Delay33/1
  Delay32/1 -> Relational1/2
  Delay35/1 -> snap_sync_gen/13(trig)
  Delay36/1 -> snap_sync_gen/14(stop)
  From114/1 -> Delay36/1
  Logical13/1 -> snap_sync_gen/12(we)
  Delay33/1 -> Logical13/2
  Relational1/1 -> Logical13/1
  From66/1 -> Delay46/1
  [cnt_rst] -> Subsystem2/1(rst)
  [synced] -> Delay38/1
  [sync_armed] -> Delay39/1
  From29/1 -> Delay45/1
  From62/1 -> Delay44/1
  From64/1 -> Delay42/1
  From55/1 -> Delay41/1
  From57/1 -> Delay40/1
  From58/1 -> Delay37/1
  Delay37/1 -> snap_sync_gen/11(in_ct_err)
  Delay40/1 -> snap_sync_gen/10(in_cd_err)
  Delay41/1 -> snap_sync_gen/9(in_timestep_err)
  Delay42/1 -> snap_sync_gen/8(in_time_diff_err)
  Delay44/1 -> snap_sync_gen/7(in_sync_armed)
  Delay45/1 -> snap_sync_gen/6(in_synced)
  Delay46/1 -> snap_sync_gen/5(in_time)
  [up_timestep_error] -> Logical15/1
  [sys_rst] -> Logical9/1
  Logical9/1 -> edge_detect17/1(in)
  [time_diff_error] -> Logical15/4
  [cd_error] -> Logical15/2
  [ct_error] -> Logical15/3
  edge_detect17/1(out) -> [sys_relock], Register/2
  [pack_sync] -> Register/3, Register/1
  Counter3/1 -> Slice13/1
  Slice13/1 -> edge_detect8/1(in)
  Logical15/1 -> [fault_detected]
  Register6/1 -> Inverter2/1
  Register/1 -> posedge_delay1/1(In1), [synced], posedge_delay/1(In1)
  posedge_delay/1(Out1) -> [synced_delay]
  [board_in_fault] -> Delay48/1
  Delay49/1 -> snap_sync_gen/4(in_board_in_fault)
  From198/1 -> Delay49/1
  [synced] -> Inverter1/1
  Inverter1/1 -> Counter1/2
  [pack_sync] -> Counter1/1
  Counter1/1 -> Slice16/1
  Slice16/1 -> edge_detect7/1(in)
  [q_sync] -> Subsystem19/5(in3)
  [pfb_sync] -> Subsystem19/3(in1)
  [fdfs_sync] -> Subsystem19/4(in2)
  [sync80] -> Subsystem19/2(in0)
  [cnt_rst] -> Subsystem19/1(rst)
  Subsystem19/2(out1) -> sync_status2/2(out_sync_pfb_cnt)
  Subsystem19/1(out0) -> sync_status2/1(out_sync80_cnt)
  Subsystem19/3(out2) -> sync_status2/3(out_sync_fdfs_cnt)
  Subsystem19/4(out3) -> sync_status2/4(out_sync_quant_cnt)
  [pack_sync] -> Subsystem9/4(in2)
  [flag_sync] -> Subsystem9/3(in1)
  [ct_sync] -> Subsystem9/2(in0)
  [cnt_rst] -> Subsystem9/1(rst)
  [resync_allow] -> Subsystem2/2(armed)
  [sync_timeout] -> Subsystem2/3(in1)
  [time_diff_error] -> Subsystem2/4(in2)
  [up_timestep_error] -> Subsystem2/5(in3)
  [cd_error] -> Subsystem2/6(in4)
  [ct_error] -> Subsystem2/7(in5)
  Delay48/1 -> sync_status0/2(out_board_in_fault)
  Delay38/1 -> sync_status0/3(out_synced)
  Delay39/1 -> sync_status0/4(out_sync_armed)
  Subsystem9/1(out0) -> sync_status0/5(out_sync_ct)
  Subsystem9/2(out1) -> sync_status0/6(out_sync_flag)
  Subsystem9/3(out2) -> sync_status0/7(out_sync_pack)
  From204/1 -> Delay54/1
  From207/1 -> Delay55/1
  Delay54/1 -> snap_sync_gen/3(in_pack_sync)
  Delay55/1 -> snap_sync_gen/2(in_sync_timeout)
  Subsystem2/5(Out5) -> sync_status1/5(out_ct_resync_cnt)
  Subsystem2/1(Out1) -> sync_status1/1(out_timeout_resync_cnt)
  Subsystem2/2(Out2) -> sync_status1/2(out_time_diff_resync_cnt)
  Subsystem2/3(Out3) -> sync_status1/3(out_timestep_resync_cnt)
  Subsystem2/4(Out4) -> sync_status1/4(out_cd_resync_cnt)
  From206/1 -> Delay56/1
  Delay56/1 -> snap_sync_gen/1(in_synced_delay)
  [sys_relock] -> Delay57/1
  Inverter2/1 -> [board_in_fault]
  Delay57/1 -> Register6/2
  [synced_delay] -> edge_detect9/1(in)
  edge_detect9/1(out) -> Register6/3, Register6/1
  [synced_delay] -> Delay58/1
  Delay58/1 -> sync_status0/1(out_synced_delay)
  edge_detect7/1(out) -> [sync_timeout]
  [auto_rst_enable] -> Logical8/1
  [resync_allow] -> Logical8/2
  [fault_detected] -> Logical8/3
  [auto_rst_enable] -> Logical14/1
  Logical14/1 -> Logical9/2
  Logical8/1 -> Logical9/3
  [fault_detected] -> Counter5/1
  Counter5/1 -> Slice20/1
  Slice20/1 -> edge_detect10/1(in), Inverter3/1
  Inverter3/1 -> Counter5/2
  [fault_detected] -> Counter3/1
  edge_detect10/1(out) -> [fault_clear_timeout]
  [sync_timeout] -> Logical10/1
  [fault_clear_timeout] -> Logical10/2
  Logical10/1 -> Logical14/2
  edge_detect8/1(out) -> [fault_present_timeout]
  [fault_present_timeout] -> Logical10/3
  posedge_delay1/1(Out1) -> [resync_allow]
  Subsystem2/6(Out6) -> sync_status1/6(out_fault_clear_timeout_cnt)
  Subsystem2/7(Out7) -> sync_status1/7(out_fault_present_timeout_cnt)
  [fault_clear_timeout] -> Subsystem2/8(in6)
  [fault_present_timeout] -> Subsystem2/9(in7)
  Constant3/1 -> Relational4/1
  Relational4/1 -> Logical2/1
  Relational2/1 -> Logical2/2
  Logical2/1 -> Logical/1
  Concat5/1 -> time_gen_cd/6(rd_misc_in)
  time_gen_cd/4(rd_misc_out) -> bus_expand2/1(bus_in)
  [sync_tl_cd0] -> time_gen_cd/1(wr_sync_in)
  [dvalid_tl_cd0] -> time_gen_cd/2(wr_en)
  [hmc_sync_p0] -> time_gen_cd/4(rd_sync_in)
  [hmc_dvalid] -> time_gen_cd/5(rd_en)
  time_gen_cd/1(rd_sync_out) -> [tg_rd_sync]
  time_gen_cd/2(rd_dvalid) -> [tg_rd_dvalid]
  [time80_tl_cd0] -> Slice9/1
  Slice9/1 -> time_gen_cd/3(wr_val_in)
  Constant35/1 -> Concat7/2
  time_gen_cd/3(rd_val_out) -> Concat7/1
  Concat7/1 -> [tg_rd_time_out]
  [hmc_data_p0] -> Concat5/1
  [hmc_data_p1] -> Concat5/2
  bus_expand2/1(msb_out2) -> [tg_data_p0]
  bus_expand2/2(lsb_out1) -> [tg_data_p1]
  [hmc_dvalid] -> Subsystem26/1(In1)
  [dvalid_tl_cd0] -> Subsystem25/1(In1)
  trig_time_msw/1(in_msw) -> pipeline28/1(d)
  trig_time_lsw/1(in_lsw) -> pipeline44/1(d)
  Concat13/1 -> Relational10/1
  pipeline28/1(q) -> Concat13/1
  pipeline44/1(q) -> Concat13/2
  [time80_48] -> Relational10/2
  pipeline57/1(q) -> bus_expand7/1(bus_in)
  [d80_adc1] -> pipeline163/1(d)
  [valid80] -> Slice5/1
  Slice14/1 -> pipeline162/1(d)
  [time80_48] -> Slice14/1
  pipeline162/1(q) -> snap_adc0/14(extra_timestamp)
  Slice5/1 -> pipeline161/1(d)
  [d80_adc0] -> pipeline57/1(d)
  bus_expand7/4(out5) -> snap_adc0/4(in_p0_d3)
  bus_expand7/5(out4) -> snap_adc0/5(in_p0_d4)
  bus_expand7/1(msb_out8) -> snap_adc0/1(in_p0_d0)
  bus_expand7/2(out7) -> snap_adc0/2(in_p0_d1)
  bus_expand7/3(out6) -> snap_adc0/3(in_p0_d2)
  bus_expand7/6(out3) -> snap_adc0/6(in_p0_d5)
  bus_expand7/7(out2) -> snap_adc0/7(in_p0_d6)
  bus_expand7/8(lsb_out1) -> snap_adc0/8(in_p0_d7)
  pipeline161/1(q) -> snap_adc0/9(in_dv), snap_adc0/11(we)
  Relational10/1 -> Logical12/1
  [valid80] -> pipeline126/1(d)
  Logical12/1 -> snap_adc1/10(trig), snap_adc0/12(trig)
  pipeline163/1(q) -> bus_expand1/1(bus_in)
  bus_expand1/3(out6) -> snap_adc1/3(in_p1_d2)
  bus_expand1/4(out5) -> snap_adc1/4(in_p1_d3)
  bus_expand1/2(out7) -> snap_adc1/2(in_p1_d1)
  bus_expand1/1(msb_out8) -> snap_adc1/1(in_p1_d0)
  bus_expand1/5(out4) -> snap_adc1/5(in_p1_d4)
  bus_expand1/6(out3) -> snap_adc1/6(in_p1_d5)
  bus_expand1/7(out2) -> snap_adc1/7(in_p1_d6)
  bus_expand1/8(lsb_out1) -> snap_adc1/8(in_p1_d7)
  [valid80] -> Slice1/1
  Slice1/1 -> pipeline30/1(d)
  pipeline30/1(q) -> snap_adc1/9(we)
  Slice10/1 -> pipeline32/1(d)
  [time80_48] -> Slice10/1
  pipeline32/1(q) -> snap_adc1/12(extra_timestamp)
  pipeline126/1(q) -> Logical12/2
  Delay98/1 -> adc_trig/1(adc_data_p0)
  [d80_adc0] -> Delay98/1
  adc_trig/1(trig) -> Delay105/1
  trig_level/1(in_level) -> Delay100/1
  Delay105/1 -> snap_adc1/11(stop), snap_adc0/13(stop)
  Delay100/1 -> adc_trig/3(trig_pnt)
  [d80_adc1] -> Delay99/1
  Delay99/1 -> adc_trig/2(adc_data_p1)
  [flag_dvalid] -> Subsystem13/1(In1)
  Subsystem13/1(Out1) -> pack_in_dv_rate/1(out_dv_rate)
  [s256_v] -> Subsystem11/1(In1)
  Subsystem11/1(Out1) -> pack_out_dv_rate/1(out_dv_rate)
  pipeline121/1(q) -> Convert/1
  pipeline124/1(q) -> [ip_per_x]
  pipeline125/1(q) -> [num_x]
  x_setup/1(in_f_per_x) -> pipeline121/1(d)
  x_setup/2(in_ip_per_x) -> pipeline124/1(d)
  x_setup/3(in_num_x) -> pipeline125/1(d)
  pipeline120/1(q) -> [pack_snap_arm]
  x_setup/4(in_snap_arm) -> pipeline120/1(d)
  pipeline130/1(q) -> [pktstart_sel]
  x_setup/5(in_pktstart_mux) -> pipeline130/1(d)
  [s256_v] -> pack_block_check/1(dv)
  [cnt_rst] -> Subsystem14/1(rst)
  Subsystem14/1(out0) -> pack_dv_err/1(out_dvblock_err_cnt)
  pack_block_check/1(error) -> [pack_dv_err], Subsystem14/2(in0)
  pipeline149/1(q) -> [pack_mux]
  x_setup/6(in_pack_mux) -> pipeline149/1(d)
  Convert/1 -> [f_per_x]
  x_setup/7(in_pktoffset_sel) -> pipeline63/1(d)
  pipeline63/1(q) -> [pktoffset_sel]
  iptx_base/1(in_reg) -> pipeline105/1(d)
  pipeline105/1(q) -> [tx_ip_base]
  tx_metadata/1(in_porttx) -> pipeline106/1(d)
  tx_metadata/2(in_board_id) -> pipeline107/1(d)
  pipeline106/1(q) -> [tx_port]
  pipeline107/1(q) -> [tx_board_id]
  pipeline17/1(q) -> [outfreq_stopmux]
  ct_debug/6(in_outfreq_stopmux) -> pipeline17/1(d)
  pipeline18/1(q) -> [out_stopmux]
  ct_debug/5(in_out_stopmux) -> pipeline18/1(d)
  pipeline55/1(q) -> [wrrd_stopmux]
  ct_debug/3(in_wrrd_stopmux) -> pipeline55/1(d)
  pipeline56/1(q) -> [in_stopmux]
  ct_debug/1(in_in_stopmux) -> pipeline56/1(d)
  pipeline122/1(q) -> [ct_snap_arm]
  pipeline147/1(q) -> edge_detect5/1(in)
  ct_debug/8(in_snap_trig) -> pipeline147/1(d)
  ct_debug/7(in_snap_arm) -> pipeline122/1(d)
  edge_detect5/1(out) -> [ct_snap_trig]
  ct_debug/2(in_in_trigmux) -> pipeline150/1(d)
  pipeline150/1(q) -> [in_trigmux]
  ct_debug/4(in_obuf_stopmux) -> pipeline167/1(d)
  pipeline167/1(q) -> [obuf_stopmux]
  ct_debug/9(in_snap_wesel) -> pipeline8/1(d)
  pipeline8/1(q) -> [ct_snap_wesel]
  pipeline157/1(q) -> [ct_snap_trigsel]
  ct_debug/10(in_snap_trigsel) -> pipeline157/1(d)
  pipeline166/1(q) -> [ct_snap_circsel]
  ct_debug/11(in_snap_circsel) -> pipeline166/1(d)
  [flag_sync] -> packetiser/1(sync_in)
  [flag_dvalid] -> packetiser/2(en)
  [flag_pktstart] -> packetiser/5(pkt_start)
  [flag_pktxoffset] -> packetiser/7(pkt_x_offset)
  [tx_ip_base] -> packetiser/9(base_ip)
  [tx_port] -> packetiser/10(base_port)
  Constant28/1 -> concat1/2
  [flag_time] -> concat1/1
  [flag_misc] -> packetiser/3(din)
  concat1/1 -> [pack_sync_time], packetiser/4(timestamp)
  Delay82/1 -> [s256_d]
  Delay83/1 -> [s256_v]
  Delay84/1 -> [s256_eof]
  Delay85/1 -> [s256_of]
  Delay86/1 -> [s256_ip]
  Delay87/1 -> [s256_port]
  Delay88/1 -> [pack_sync]
  packetiser/1(dout) -> Delay82/1
  packetiser/2(dvalid) -> Delay83/1
  packetiser/3(eof) -> Delay84/1
  packetiser/4(overflow) -> Delay85/1
  packetiser/5(destination_ip) -> Delay86/1
  packetiser/6(destination_port) -> Delay87/1
  packetiser/7(sync) -> Delay88/1
  [flag_pktfreq] -> Delay77/1
  Delay89/1 -> [s256_pktfreq]
  Delay77/1 -> Delay89/1
  [flag_pktxindex] -> Delay78/1
  Delay78/1 -> Delay90/1
  Delay90/1 -> [s256_pktxindex]
  [flag_pktxoffset] -> Delay79/1
  Delay79/1 -> Delay91/1
  Delay91/1 -> [s256_pktxoffset]
  [tx_board_id] -> packetiser/8(board_id)
  [flag_pktstart] -> Delay80/1
  Delay80/1 -> Delay92/1
  Delay92/1 -> [s256_pktstart]
  [flag_pktxindex] -> packetiser/6(pkt_x_index)
  [flag_time] -> Delay81/1
  Delay81/1 -> Delay93/1
  Delay93/1 -> [s256_time]
  bus_create2/1(bus_out) -> [tvgtone_level0]
  bus_create3/1(bus_out) -> [tvgtone_level1]
  tvg_tone_levels/2(in_p0i) -> bus_create2/2(in2)
  tvg_tone_levels/3(in_p1r) -> bus_create3/1(in1)
  tvg_tone_levels/4(in_p1i) -> bus_create3/2(in2)
  tvg_tone_levels/1(in_p0r) -> bus_create2/1(in1)
  tvg_tone_targets/1(in_p0) -> Slice18/1
  tvg_tone_targets/2(in_p1) -> Slice19/1
  we_delay49/1(q) -> [ct_tag_insert_sel]
  edge_detect3/1(out) -> [ct_rst_err_latch]
  we_delay47/1(q) -> edge_detect3/1(in)
  we_delay48/1(q) -> [ct_fake_data_error]
  we_delay13/1(q) -> [ct_tvg_en]
  we_delay50/1(q) -> [ct_tvg_en2]
  ct_control0/1(in_tvg_en) -> we_delay13/1(d)
  ct_control0/2(in_tvg_en2) -> we_delay50/1(d)
  ct_control0/3(in_rst_err_latch) -> we_delay47/1(d)
  ct_control0/4(in_fake_error) -> we_delay48/1(d)
  ct_control0/5(in_tag_insert) -> we_delay49/1(d)
  we_delay126/1(q) -> [obuf_read_gap]
  ct_control0/6(in_obuf_read_gap) -> we_delay126/1(d)
  we_delay41/1(q) -> [ct_num_xeng]
  we_delay112/1(q) -> [ct_num_xeng_recip]  "NUM_X_RECIP"
  ct_control1/2(in_num_x_recip) -> we_delay112/1(d)
  ct_control1/1(in_num_x) -> we_delay41/1(d)
  we_delay114/1(q) -> [ct_x_per_board]
  ct_control1/3(in_x_per_board) -> we_delay114/1(d)
  we_delay113/1(q) -> [ct_chans_per_board]
  ct_control2/1(in_chans_per_x) -> we_delay39/1(d)
  ct_control2/2(in_chans_per_board) -> we_delay113/1(d)
  we_delay115/1(q) -> [ct_x_per_board_recip]
  ct_control1/4(in_x_per_board_recip) -> we_delay115/1(d)
  we_delay38/1(q) -> [ct_num_x_boards]
  ct_control3/1(in_num_x_boards) -> we_delay38/1(d)
  we_delay37/1(q) -> [ct_num_x_boards_recip]
  ct_control3/2(in_num_x_boards_recip) -> we_delay37/1(d)
  Slice18/1 -> [tvgtone_p0]
  Slice19/1 -> [tvgtone_p1]
  Slice36/1 -> we_delay116/1(d)
  ct_control4/1(in_ct_board_offset) -> Slice36/1
  ct_control5/1(in_ct_freq_gen_offset) -> we_delay117/1(d)
  we_delay116/1(q) -> [ct_board_hmc_offset]
  we_delay117/1(q) -> [ct_freq_gen_offset]
  we_delay39/1(q) -> [ct_chans_per_x]  "PER_X"
  pipeline140/1(q) -> Counter15/1
  pipeline141/1(q) -> Counter15/2
  pipeline142/1(q) -> Counter7/1
  pipeline144/1(q) -> Counter7/2
  pipeline145/1(q) -> Counter6/2
  pipeline146/1(q) -> Counter6/1
  quant_snap_ctrl/1(in_single_channel) -> [quant_snap_single_channel]
  quant_snap_ctrl/2(in_channel_select) -> Slice3/1
  Subsystem26/1(Out1) -> cd_out_dv_rate/1(out_reg)
  Subsystem25/1(Out1) -> cd_in_dv_rate/1(out_reg)
  pipeline209/1(q) -> time_gen_nb/3(wr_val_in)
  Delay9/1 -> pipeline202/1(d), AddSub/1, Register1/1
  Delay11/1 -> pipeline203/1(d), AddSub/2, Register3/1
  From323/1 -> edge_detect11/1(in), pipeline205/1(d)
  edge_detect11/1(out) -> pipeline206/1(d)
  pipeline202/1(q) -> snap_time_check/1(in_time80_48)
  pipeline203/1(q) -> snap_time_check/2(in_pack_sync_time)
  pipeline204/1(q) -> snap_time_check/3(in_time_diff)
  pipeline205/1(q) -> snap_time_check/4(we)
  pipeline206/1(q) -> snap_time_check/5(trig)
  [sync80] -> pipeline213/1(d)
  pipeline213/1(q) -> snap_adc0/10(in_sync)
  [time80_48] -> pipeline209/1(d)
  From337/1 -> pipeline230/1(d)
  pipeline229/1(q) -> Counter12/2
  pipeline230/1(q) -> Counter12/1
  From336/1 -> Logical17/1
  From339/1 -> Logical17/2
  Logical17/1 -> pipeline229/1(d)
  Counter15/1 -> pipeline94/1(d)
  Counter6/1 -> pipeline95/1(d)
  Counter12/1 -> pipeline109/1(d)
  Counter7/1 -> pipeline117/1(d)
  pipeline94/1(q) -> ddc_status/1(out_in_sync_cnt)
  pipeline95/1(q) -> ddc_status/2(out_out_sync_cnt)
  pipeline109/1(q) -> ddc_status/3(out_out_sync_cnt1)
  pipeline117/1(q) -> ddc_status/4(out_dv_cnt)
  tl_fd1/3(sync_out) -> fd_nb1/1(sync_in)
  tl_fd1/4(dout) -> fd_nb1/2(din)
  tl_fd1/5(dvalid) -> fd_nb1/3(en)
  tl_fd1/2(enable) -> fd_nb1/5(load_value)
  tl_fd1/1(value) -> fd_nb1/4(delay_value)
  [d80_adc0] -> Delay96/1
  [d80_adc1] -> Delay97/1
  calc_adc_sum_sq0/1(mean_pwr) -> Delay94/1
  Delay94/1 -> adc_pwr0/1(out_reg)
  Delay95/1 -> adc_pwr1/1(out_reg)
  Delay96/1 -> calc_adc_sum_sq0/1(adc_in)
  Delay97/1 -> calc_adc_sum_sq1/1(adc_in)
  calc_adc_sum_sq1/1(mean_pwr) -> Delay95/1
  Delay102/1 -> adc_dev0/1(out_max)
  Delay101/1 -> adc_dev0/2(out_min)
  calc_adc_sum_sq0/2(max) -> Delay102/1
  calc_adc_sum_sq0/3(min) -> Delay101/1
  Delay104/1 -> adc_dev1/1(out_max)
  Delay103/1 -> adc_dev1/2(out_min)
  calc_adc_sum_sq1/2(max) -> Delay104/1
  calc_adc_sum_sq1/3(min) -> Delay103/1
  [q_d64_0] -> Delay116/1
  [q_d64_1] -> Delay117/1
  calc_quant_pwr0/1(mean_pwr) -> pipeline160/1(d)
  calc_quant_pwr1/1(mean_pwr) -> pipeline165/1(d)
  Delay116/1 -> calc_quant_pwr0/1(adc_in)
  Delay117/1 -> calc_quant_pwr1/1(adc_in)
  pipeline160/1(q) -> quant_pwr0/1(out_reg)
  pipeline165/1(q) -> quant_pwr1/1(out_reg)
  [q_dv] -> Delay114/1
  Delay114/1 -> calc_quant_pwr0/2(valid_in)
  [q_dv] -> Delay115/1
  Delay115/1 -> calc_quant_pwr1/2(valid_in)
  bus_expand3/8(lsb_out1) -> snap_quant0/8(in_imag3)
  bus_expand3/7(out2) -> snap_quant0/7(in_real3)
  bus_expand3/6(out3) -> snap_quant0/6(in_imag2)
  bus_expand3/5(out4) -> snap_quant0/5(in_real2)
  bus_expand3/3(out6) -> snap_quant0/3(in_real1)
  bus_expand3/4(out5) -> snap_quant0/4(in_imag1)
  bus_expand3/1(msb_out8) -> snap_quant0/1(in_real0)
  bus_expand3/2(out7) -> snap_quant0/2(in_imag0)
  quant_snap_filter0/1(data_valid_out) -> snap_quant0/9(we)
  quant_snap_filter0/3(packet_sync_out) -> snap_quant0/10(trig)
  pipeline267/1(q) -> ddc_status1/2(out_ddc_of1)
  pipeline266/1(q) -> ddc_status1/1(out_ddc_of0)
  Counter19/1 -> pipeline266/1(d)
  Counter20/1 -> pipeline267/1(d)
  [cnt_rst] -> pipeline268/1(d)
  pipeline269/1(q) -> Counter19/2
  pipeline268/1(q) -> pipeline270/1(d), Counter19/1
  pipeline271/1(q) -> Counter20/2
  DDC/5(ddc_of) -> [ddc_of]
  [ddc_of] -> bus_expand12/1(bus_in)
  bus_expand12/1(msb_out2) -> pipeline269/1(d)
  bus_expand12/2(lsb_out1) -> pipeline271/1(d)
  Concat16/1 -> time_gen_4/6(rd_misc_in)
  [sync80] -> time_gen_4/1(wr_sync_in)
  [valid80] -> time_gen_4/2(wr_en)
  [pfbin_sync] -> time_gen_4/4(rd_sync_in)
  [pfbin_dv] -> time_gen_4/5(rd_en)
  time_gen_4/3(rd_val_out) -> [tg_dds_time_out]
  [pfbin_d0] -> Concat16/1
  [pfbin_d1] -> Concat16/2
  bus_expand13/1(msb_out2) -> [tg_dds_data_p0]
  bus_expand13/2(lsb_out1) -> [tg_dds_data_p1]
  ct_control0/7(in_chans_per_x_recip) -> we_delay124/1(d)
  we_delay124/1(q) -> [ct_chans_per_x_recip]
  [tg_dds_data_p0] -> complexify/1(In1)
  [tg_dds_sync] -> Concat17/1
  [tg_dds_dvalid] -> Concat17/2
  complexify/1(Out1) -> Concat17/3
  Constant74/1 -> freq_cwg_osc/1(sim_1)
  freq_cwg_osc/1(in_frequency) -> [osc_freq]
  [osc_cmplx] -> DDC/6(osc1), DDC/4(osc0)
  pipeline290/1(q) -> pfb_status1/2(out_pol1_err_cnt)
  Subsystem5/2(out1) -> pipeline225/1(d)
  pipeline287/1(q) -> Counter21/2
  pipeline286/1(q) -> Counter21/1
  [pfb_data_out_0] -> Delay112/1
  nb_pfb/1(sync_out) -> Delay127/1
  Delay106/1 -> calc_fft_pwr0/2(valid_in)
  calc_fft_pwr1/1(mean_pwr) -> pfb_pwr1/1(out_scale8)
  Counter25/1 -> pipeline292/1(d)
  Relational5/1 -> Counter23/2
  pipeline153/1(q) -> Counter8/2
  [pfb_of] -> Slice22/1, Slice21/1
  pipeline289/1(q) -> Counter22/2
  pipeline288/1(q) -> Counter22/1
  [cnt_rst] -> Counter25/1, Counter24/1, Counter23/1
  pipeline154/1(q) -> Counter8/1
  Delay112/1 -> calc_fft_pwr0/1(adc_in)
  [pfb_data_out_1] -> Delay107/1
  Delay107/1 -> calc_fft_pwr1/1(adc_in)
  [pfb_dv] -> Delay110/1
  pipeline119/1(q) -> nb_status/2(out_out_sync_cnt1)
  pipeline293/1(q) -> pfb_status/5(out_p0_fifo_full_cnt)
  [pfb_dv] -> Delay106/1
  Counter22/1 -> pipeline290/1(d)
  pipeline291/1(q) -> pfb_status1/1(out_pol0_err_cnt)
  fft_shift_munge/1(dout) -> pipeline295/1(d)
  Slice22/1 -> Subsystem5/2(in0)
  calc_fft_pwr0/1(mean_pwr) -> pfb_pwr0/1(out_scale8)
  pipeline118/1(q) -> nb_status/1(out_out_sync_cnt)
  Constant67/1 -> fft_shift/1(sim_1)
  [pfb_sync] -> pipeline153/1(d)
  nb_pfb/2(dv_out) -> Delay128/1
  pipeline159/1(q) -> nb_status/3(out_dv_cnt)
  pipeline152/1(q) -> Counter9/1
  [pfb_dv] -> Logical16/2
  [cnt_rst] -> pipeline285/1(d)
  Delay110/1 -> calc_fft_pwr1/2(valid_in)
  nb_pfb/4(pol1_out) -> Delay131/1
  [fft_shift] -> nb_pfb/5(fft_shift)
  Counter10/1 -> pipeline119/1(d)
  [cnt_rst] -> pipeline154/1(d)
  [pfb_sync] -> Logical16/1
  [pfb_dv] -> pipeline151/1(d)
  Counter24/1 -> pipeline293/1(d)
  [cnt_rst] -> pipeline152/1(d)
  pipeline285/1(q) -> Counter10/1
  nb_pfb/5(pfb_of) -> Delay133/1
  fft_shift/1(in_fft_shift) -> fft_shift_munge/1(din)
  pipeline284/1(q) -> Counter10/2
  nb_pfb/3(pol0_out) -> Delay130/1
  Logical16/1 -> pipeline284/1(d)
  Counter8/1 -> pipeline118/1(d)
  [clr_status] -> Subsystem5/1(rst)
  pipeline295/1(q) -> [fft_shift]
  [fft_pol1_err] -> pipeline289/1(d)
  Subsystem5/1(out0) -> pipeline226/1(d)
  Counter23/1 -> pipeline294/1(d)
  pipeline226/1(q) -> pfb_status/1(out_pol0_or_err_cnt)
  [fft_ch1] -> Relational5/2
  [cnt_rst] -> pipeline286/1(d)
  [fft_p1_fifo_full] -> Counter25/2
  [cnt_rst] -> pipeline288/1(d)
  [pfb_sync] -> Subsystem5/4(in2)
  Slice21/1 -> Subsystem5/3(in1)
  pipeline294/1(q) -> pfb_status/4(out_fft_ch_diff_cnt)
  Counter9/1 -> pipeline159/1(d)
  [fft_p0_fifo_full] -> Counter24/2
  [fft_pol0_err] -> pipeline287/1(d)
  [fft_ch0] -> Relational5/1
  pipeline292/1(q) -> pfb_status/6(out_p1_fifo_full_cnt)
  pipeline151/1(q) -> Counter9/2
  Subsystem5/3(out2) -> pipeline85/1(d)
  pipeline225/1(q) -> pfb_status/2(out_pol1_or_err_cnt)
  pipeline85/1(q) -> pfb_status/3(out_sync_cnt)
  Counter21/1 -> pipeline291/1(d)
  Delay123/1 -> Concat11/2
  Constant78/1 -> delta_delay0/1(sim_1)
  Delay121/1 -> pipeline172/1(d)
  Constant41/1 -> delay_frac1/1(sim_1)
  phase0/1(in_initial) -> Reinterpret2/1
  pipeline135/1(q) -> [tl_delay0_load_immediate]
  pipeline174/1(q) -> Concat14/2
  Constant60/1 -> Delay122/1
  Concat14/1 -> [ld_val1]
  Concat11/1 -> pipeline169/1(d)
  Concat3/1 -> pipeline173/1(d)
  delay1_tl_control0/3(in_load_time_msw) -> Concat8/1
  Concat8/1 -> pipeline143/1(d)
  Reinterpret9/1 -> Delay124/1
  delay_whole1/1(in_initial) -> Reinterpret4/1
  delay0_tl_control0/1(in_arm) -> pipeline134/1(d)
  Constant12/1 -> delay_whole0/1(sim_1)
  pipeline134/1(q) -> [tl_delay0_arm]
  phase1/1(in_initial) -> Reinterpret9/1
  pipeline138/1(q) -> [tl_delay1_load_immediate]
  pipeline170/1(q) -> Concat22/2
  Constant43/1 -> delay0_tl_control0/3(sim_3)
  Constant62/1 -> phase1/1(sim_1)
  pipeline137/1(q) -> [tl_delay1_arm]
  Constant61/1 -> delay_whole1/1(sim_1)
  delay0_tl_control0/2(in_load_immediate) -> pipeline135/1(d)
  pipeline171/1(q) -> Concat22/3
  Constant46/1 -> delay0_tl_control1/1(sim_1)
  phase_rate1/1(in_delta) -> Reinterpret12/1
  Constant57/1 -> delay1_tl_control1/1(sim_1)
  pipeline173/1(q) -> Concat14/1
  delay0_tl_control1/1(in_load_time_lsw) -> Concat6/2
  Constant40/1 -> delta_delay1/1(sim_1)
  Delay124/1 -> pipeline175/1(d)
  delta_delay0/1(in_initial) -> Reinterpret20/1
  Delay119/1 -> pipeline174/1(d)
  Constant76/1 -> delay_frac0/1(sim_1)
  Constant75/1 -> phase_rate0/1(sim_1)
  delay0_tl_control0/3(in_load_time_msw) -> Concat6/1
  Reinterpret12/1 -> Delay125/1
  Delay125/1 -> pipeline176/1(d)
  Constant55/1 -> delay1_tl_control0/2(sim_2)
  Delay126/1 -> Concat3/1
  Constant10/1 -> phase0/1(sim_1)
  pipeline175/1(q) -> Concat14/3
  Delay113/1 -> delay0_tl_control0/1(sim_1)
  Concat22/1 -> [ld_val0]
  Delay120/1 -> pipeline171/1(d)
  Reinterpret1/1 -> Delay12/1
  pipeline136/1(q) -> [tl_delay0_load_time]
  pipeline176/1(q) -> Concat14/4
  pipeline169/1(q) -> Concat22/1
  Delay12/1 -> Concat3/2
  delay_frac0/1(in_initial) -> Reinterpret18/1
  Reinterpret2/1 -> Delay120/1
  phase_rate0/1(in_delta) -> Reinterpret3/1
  Constant45/1 -> delay0_tl_control0/2(sim_2)
  delay1_tl_control0/1(in_arm) -> pipeline137/1(d)
  delay_frac1/1(in_initial) -> Reinterpret1/1
  Reinterpret4/1 -> Delay126/1
  Reinterpret3/1 -> Delay121/1
  Constant48/1 -> delay1_tl_control0/3(sim_3)
  Reinterpret19/1 -> Delay118/1
  Constant47/1 -> Delay113/1
  Concat6/1 -> pipeline136/1(d)
  Delay13/1 -> pipeline170/1(d)
  delta_delay1/1(in_initial) -> Reinterpret5/1
  Reinterpret18/1 -> Delay123/1
  delay1_tl_control0/2(in_load_immediate) -> pipeline138/1(d)
  Reinterpret20/1 -> Delay13/1
  delay_whole0/1(in_initial) -> Reinterpret19/1
  delay1_tl_control1/1(in_load_time_lsw) -> Concat8/2
  Delay118/1 -> Concat11/1
  Constant42/1 -> phase_rate1/1(sim_1)
  Delay122/1 -> delay1_tl_control0/1(sim_1)
  pipeline143/1(q) -> [tl_delay1_load_time]
  Reinterpret5/1 -> Delay119/1
  pipeline172/1(q) -> Concat22/4
  [d80_adc0] -> pipeline71/1(d)
  bs_delay1/2(data_out) -> [delay_d1]
  [delay_tl_bs0] -> bs_delay0/2(delay_val)
  [delay_tl_sync0] -> bs_delay0/1(sync)
  pipeline92/1(q) -> tl_cd0/10(load_time)
  Constant34/1 -> tl_bs0/7(misci)
  tl_bs0/2(enable) -> [en_tl_bs0]
  [tl_delay1_load_time] -> tl_bs1/10(load_time)
  [tl_delay0_load_immediate] -> tl_bs0/9(load_immediate)
  tl_bs1/4(dout) -> [data_tl_bs1]
  [clr_status] -> tl_bs1/1(cnt_rst)
  [clr_status] -> pipeline25/1(d), pipeline75/1(d)
  tl_cd1/3(sync_out) -> [sync_tl_cd1]
  tl_bs1/7(misco) -> Terminator10/1
  [tg_rd_dvalid] -> tl_bs1/6(en)
  tl_cd1/6(time) -> [time80_tl_cd1]
  [dvalid_tl_bs0] -> bs_delay0/4(en)
  [ld_val1] -> pipeline26/1(d)
  [tl_delay0_load_time] -> pipeline92/1(d)
  bs_delay0/2(data_out) -> [delay_d0]
  [tl_delay1_arm] -> tl_bs1/8(arm)
  pipeline24/1(q) -> tl_cd1/2(current_time)
  [tl_delay1_load_immediate] -> tl_bs1/9(load_immediate)
  pipeline76/1(q) -> tl_cd0/6(en)
  [tl_delay1_load_time] -> pipeline40/1(d)
  Gateway Out7/1 -> To Workspace7/1
  pipeline25/1(q) -> tl_cd1/1(cnt_rst)
  [d80_adc1] -> pipeline33/1(d)
  [tg_data_p1] -> tl_bs1/5(din)
  [dvalid_tl_bs1] -> bs_delay1/4(en)
  bs_delay1/3(dvalid) -> Terminator11/1
  [tl_delay0_arm] -> tl_bs0/8(arm)
  [tg_rd_sync] -> tl_bs0/4(sync_in)
  [valid80] -> pipeline34/1(d), pipeline76/1(d)
  tl_cd0/6(time) -> [time80_tl_cd0]
  [en_tl_bs0] -> bs_delay0/5(load_val)
  tl_bs0/5(dvalid) -> [dvalid_tl_bs0]
  [tl_delay0_load_time] -> tl_bs0/10(load_time)
  pipeline75/1(q) -> tl_cd0/1(cnt_rst)
  tl_bs0/4(dout) -> [data_tl_bs0]
  tl_bs0/6(time) -> Terminator13/1
  pipeline91/1(q) -> tl_cd0/9(load_immediate)
  tl_cd1/1(value) -> [delay_tl_cd1]
  [tg_rd_time_out] -> tl_bs0/2(current_time)
  pipeline40/1(q) -> tl_cd1/10(load_time)
  bs_delay0/1(sync_out) -> [delay_sync]
  [tg_rd_time_out] -> tl_bs1/2(current_time)
  [ld_val0] -> pipeline73/1(d)
  tl_bs1/5(dvalid) -> [dvalid_tl_bs1]
  [delay_tl_bs1] -> bs_delay1/2(delay_val)
  pipeline73/1(q) -> tl_cd0/3(load_value)
  tl_bs0/3(sync_out) -> [delay_tl_sync0]
  [ld_val1] -> tl_bs1/3(load_value)
  Constant36/1 -> tl_bs1/7(misci)
  pipeline72/1(q) -> tl_cd0/4(sync_in)
  [tl_delay0_arm] -> pipeline90/1(d)
  pipeline71/1(q) -> tl_cd0/5(din)
  bs_delay0/3(dvalid) -> [delay_dv]
  tl_cd1/4(dout) -> [dout_tl_cd1]
  bs_delay1/1(sync_out) -> Terminator16/1
  Constant16/1 -> tl_cd0/7(misci)
  [data_tl_bs0] -> bs_delay0/3(din)
  tl_cd0/3(sync_out) -> [sync_tl_cd0]
  tl_cd0/4(dout) -> [dout_tl_cd0]
  pipeline74/1(q) -> tl_cd0/2(current_time)
  [tg_data_p0] -> tl_bs0/5(din)
  tl_cd0/1(value) -> [delay_tl_cd0]
  pipeline90/1(q) -> tl_cd0/8(arm)
  tl_bs0/1(value) -> [delay_tl_bs0]
  [tl_delay0_load_immediate] -> pipeline91/1(d)
  [tl_delay1_arm] -> pipeline35/1(d)
  tl_bs1/6(time) -> Terminator7/1
  tl_bs0/7(misco) -> Terminator12/1
  pipeline34/1(q) -> tl_cd1/6(en)
  [data_tl_bs1] -> bs_delay1/3(din)
  pipeline35/1(q) -> tl_cd1/8(arm)
  [tg_rd_sync] -> tl_bs1/4(sync_in)
  tl_cd0/5(dvalid) -> [dvalid_tl_cd0]
  [ld_val0] -> tl_bs0/3(load_value)
  [time80] -> pipeline24/1(d), Gateway Out7/1, pipeline74/1(d)
  [tg_rd_dvalid] -> tl_bs0/6(en)
  [delay_tl_sync1] -> bs_delay1/1(sync)
  tl_bs1/3(sync_out) -> [delay_tl_sync1]
  tl_bs1/1(value) -> [delay_tl_bs1]
  Constant17/1 -> tl_cd1/7(misci)
  tl_cd1/7(misco) -> Terminator1/1
  [en_tl_bs1] -> bs_delay1/5(load_val)
  Delay8/1 -> [hmc_sync_raw]
  [sync80] -> pipeline36/1(d), pipeline72/1(d)
  [clr_status] -> tl_bs0/1(cnt_rst)
  tl_cd0/7(misco) -> Terminator/1
  tl_cd1/2(enable) -> [en_tl_cd1]
  pipeline33/1(q) -> tl_cd1/5(din)
  pipeline37/1(q) -> tl_cd1/9(load_immediate)
  [tl_delay1_load_immediate] -> pipeline37/1(d)
  tl_cd1/5(dvalid) -> [dvalid_tl_cd1]
  pipeline26/1(q) -> tl_cd1/3(load_value)
  pipeline36/1(q) -> tl_cd1/4(sync_in)
  tl_cd0/2(enable) -> [en_tl_cd0]
  tl_bs1/2(enable) -> [en_tl_bs1]
  [tl_delay0_arm] -> tl_fd0/8(arm)
  Constant2/1 -> tl_fd0/7(misci)
  [tl_delay0_load_time] -> tl_fd0/10(load_time)
  [tl_delay0_load_immediate] -> tl_fd0/9(load_immediate)
  Constant5/1 -> tl_fd1/7(misci)
  [tl_delay1_load_immediate] -> tl_fd1/9(load_immediate)
  [tl_delay1_arm] -> tl_fd1/8(arm)
  [tl_delay1_load_time] -> tl_fd1/10(load_time)
  [ld_val1] -> tl_fd1/3(load_value)
  [tg_dds_data_p1] -> complexify2/1(In1)
  complexify2/1(Out1) -> Concat17/4
  bus_expand8/1(msb_out4) -> [ddc_sync_in]
  bus_expand8/4(lsb_out1) -> [ddc_pol1_in]
  bus_expand8/3(out2) -> [ddc_pol0_in]
  bus_expand8/2(out3) -> [ddc_dv_in]
  demux/1(sync_out) -> [fdfs_sync]
  demux/2(dv_out) -> [fdfs_dv]
  demux/3(pol0_out) -> [fdfs_d144_0]
  demux/4(pol1_out) -> [fdfs_d144_1]
  fd_nb0/1(sync_out) -> [fd_nb_sync], Gateway Out10/1, Delay143/1
  fd_nb0/3(dvalid) -> [fd_nb_dv], Gateway Out9/1, Delay142/1
  fd_nb1/2(dout) -> Delay144/1
  [tg_pfb_sync] -> tl_fd0/4(sync_in)
  [tg_pfb_sync] -> tl_fd1/4(sync_in)
  [tg_pfb_dv] -> tl_fd1/6(en)
  [tg_pfb_dv] -> tl_fd0/6(en)
  cd_hmc/3(dout1) -> sync_mangle/3(din1)
  cd_hmc/2(dout0) -> sync_mangle/2(din)
  sync_mangle/4(dvalid) -> [hmc_dvalid]
  [delay_tl_cd0] -> cd_hmc/4(delay_val)
  cd_hmc/4(dvalid) -> sync_mangle/4(en)
  cd_hmc/1(sync_out) -> Delay8/1, sync_mangle/1(sync_in)
  [dvalid_tl_cd0] -> cd_hmc/3(en)
  cd_hmc/5(hmc_error) -> [cd_error]
  sync_mangle/2(dout0) -> [hmc_data_p0]
  [dout_tl_cd0] -> cd_hmc/2(din)
  sync_mangle/1(sync_out) -> [hmc_sync_p0]
  [dvalid_tl_cd1] -> cd_hmc/8(en1)
  [sync_tl_cd0] -> cd_hmc/1(sync_in)
  sync_mangle/3(dout1) -> [hmc_data_p1]
  [dout_tl_cd1] -> cd_hmc/7(din1)
  [delay_tl_cd1] -> cd_hmc/9(delay_val1)
  [sync_tl_cd1] -> cd_hmc/6(sync_in1)
  [en_tl_cd0] -> cd_hmc/5(load_val)
  [en_tl_cd1] -> cd_hmc/10(load_val1)
  [q_dv] -> Subsystem12/1(In1)
  dv_block_check/1(error) -> [ct_dvblk_err], Subsystem6/3(in1)
  [cnt_rst] -> Subsystem6/1(rst)
  Subsystem10/4(out3) -> ct_sync_cnt/4(out_sync_out)
  pktlen_check/1(error) -> [ct_pktlen_err], Subsystem6/2(in0)
  Subsystem10/3(out2) -> ct_sync_cnt/3(out_rd_sync_cnt)
  Subsystem8/1(Out1) -> ct_out_dv_rate/1(out_reg)
  [ct_pktstart] -> pktlen_check/1(pkt_start)
  hmc_ct/3(out_d256) -> [ct_d256]
  hmc_ct/4(pkt_start) -> [ct_pktstart]
  Subsystem6/2(out1) -> ct_dv_err/2(out_dvblock_err_cnt)
  [ct_dv] -> dv_block_check/1(dv), pktlen_check/2(dv)
  hmc_ct/6(x_index) -> [ct_pkt_x_index]
  Constant9/1 -> Subsystem10/4(in2)
  [cnt_rst] -> Subsystem10/1(rst)
  Subsystem10/1(out0) -> ct_sync_cnt/1(out_sync_in)
  hmc_ct/8(error0) -> [ct_error]
  [ct_dv] -> Subsystem8/1(In1)
  Subsystem6/1(out0) -> ct_dv_err/1(out_pktlen_err_cnt)
  hmc_ct/5(freq_id) -> [ct_pktfreq]
  hmc_ct/2(out_dv) -> [ct_dv]
  Subsystem10/2(out1) -> ct_sync_cnt/2(out_rd_addr_arm_cnt)
  hmc_ct/1(out_sync) -> [ct_sync]
  hmc_ct/7(x_pkt_index) -> [ct_pkt_x_offset]
  Constant/1 -> Subsystem10/3(in1)
  [q_sync] -> Subsystem10/2(in0)
  [ct_sync] -> Subsystem10/5(in3)
  Subsystem12/1(Out1) -> ct_in_dv_rate/1(out_reg)
  [ct_tvg_en2] -> Mux1/1
  [valid80] -> time_gen1/2(wr_en)
  Delay60/1 -> Delay64/1
  Slice2/1 -> time_gen1/3(wr_val_in)
  Delay66/1 -> [flag_pktxindex]
  [ct_pkt_x_offset] -> Delay19/1
  [valid80] -> Subsystem/3(dv)
  Delay20/1 -> Delay63/1
  Delay15/1 -> Gateway Out16/1, Delay7/1
  Delay4/1 -> Gateway Out18/1, Delay5/1
  Mux1/1 -> Delay59/1  "gapvalid"
  Delay17/1 -> Mux1/2
  [ct_pktstart] -> Delay4/1
  time_gen1/1(rd_sync_out) -> [flag_sync]
  Slice4/1 -> flag_epoch_lsw/1(out_reg)
  Delay7/1 -> Delay62/1
  time_gen1/5(epoch) -> Concat10/1
  time_gen1/4(rd_misc_out) -> [flag_misc]
  Delay65/1 -> [flag_pktfreq]
  Delay5/1 -> Delay60/1
  Constant8/1 -> Concat10/2
  time_gen1/3(rd_val_out) -> [flag_time]
  time_gen1/2(rd_dvalid) -> [flag_dvalid]
  Delay62/1 -> Delay66/1
  Subsystem/1(msw) -> sync_time_msw/1(out_reg)
  [ct_pktfreq] -> Delay14/1
  Delay63/1 -> Delay67/1
  Delay16/1 -> tvg/2(dv), Delay3/1
  [time80] -> Slice2/1
  Delay6/1 -> Delay61/1
  Delay61/1 -> Delay65/1
  Slice11/1 -> flag_epoch_msw/1(out_reg)
  Delay59/1 -> time_gen1/6(rd_misc_in)
  Delay67/1 -> [flag_pktxoffset]
  Delay43/1 -> time_gen1/4(rd_sync_in)
  [ct_d256] -> Delay17/1
  [ct_pkt_x_index] -> Delay15/1
  [ct_dv] -> Delay16/1
  Delay3/1 -> Delay47/1  "gapdata"
  Delay47/1 -> time_gen1/5(rd_en)
  Concat10/1 -> Slice4/1, Slice11/1, [flag_epoch]
  Subsystem/2(ls32) -> sync_time_lsw/1(out_reg)
  Delay/1 -> Delay43/1  "gapsync"
  Delay14/1 -> Gateway Out15/1, tvg1/1(freq), Delay6/1
  [ct_sync] -> Delay18/1
  [sync80] -> Subsystem/2(sync)
  Delay18/1 -> tvg/1(sync), Delay/1
  [time80] -> Subsystem/1(time)
  Delay19/1 -> Gateway Out17/1, Delay20/1
  Delay64/1 -> [flag_pktstart]
  [sync80] -> time_gen1/1(wr_sync_in)
  From247/1 -> time_gen2/1(wr_sync_in)
  From249/1 -> time_gen2/2(wr_en)
  From_pfb_d1/1 -> time_gen2/3(wr_val_in)
  edge_detect12/1(out) -> we_delay14/1(d)
  From296/1 -> time_gen2/4(rd_sync_in)
  From297/1 -> time_gen2/5(rd_en)
  From259/1 -> Concat/1
  From267/1 -> Concat/2
  From298/1 -> Slice12/1
  Concat/1 -> time_gen2/6(rd_misc_in)
  time_gen2/3(rd_val_out) -> we_delay12/1(d)
  time_gen2/2(rd_dvalid) -> we_delay10/1(d)
  time_gen2/1(rd_sync_out) -> we_delay9/1(d), snap_ctout/9(trig), Logical11/2
  bus_expand9/3(lsb_out1) -> we_delay11/1(d)
  bus_expand9/1(msb_out3) -> Delay25/1
  bus_expand9/2(out2) -> we_delay8/1(d)
  time_gen2/4(rd_misc_out) -> bus_expand9/1(bus_in)
  we_delay1/1(q) -> sync_lat_ct/1(out_count)
  Logical11/1 -> edge_detect12/1(in)
  we_delay2/1(q) -> snap_ctout/1(in_pktstart)
  From362/1 -> time_gen3/5(rd_en)
  From361/1 -> time_gen3/4(rd_sync_in)
  From_pfb_d3/1 -> time_gen3/3(wr_val_in)
  From274/1 -> time_gen3/2(wr_en)
  From255/1 -> time_gen3/1(wr_sync_in)
  From363/1 -> Slice6/1
  Slice6/1 -> time_gen3/6(rd_misc_in)
  time_gen3/2(rd_dvalid) -> we_delay7/1(d), we_delay4/1(d)
  time_gen3/1(rd_sync_out) -> snap_qout/6(trig), we_delay3/1(d)
  time_gen3/3(rd_val_out) -> we_delay5/1(d)
  time_gen3/4(rd_misc_out) -> we_delay6/1(d)
  we_delay3/1(q) -> snap_qout/1(in_sync)
  we_delay4/1(q) -> snap_qout/2(in_dv)
  we_delay5/1(q) -> snap_qout/3(in_time)
  we_delay6/1(q) -> snap_qout/4(in_data)
  we_delay7/1(q) -> snap_qout/5(we)
  we_delay8/1(q) -> snap_ctout/2(in_freq)
  we_delay9/1(q) -> snap_ctout/3(in_sync)
  we_delay10/1(q) -> snap_ctout/4(in_dv)
  we_delay11/1(q) -> snap_ctout/5(in_data)
  we_delay12/1(q) -> snap_ctout/6(in_time)
  we_delay14/1(q) -> snap_ctout/8(we)
  Slice12/1 -> Concat/3
  [pfb_data_out_0] -> pipeline228/1(d)
  [pfb_data_out_1] -> pipeline231/1(d)
  [pfb_dv] -> pipeline212/1(d)
  [pfb_sync] -> pipeline210/1(d)
  Mux9/1 -> Goto178/1
  Mux8/1 -> Goto177/1
  Mux6/1 -> Goto175/1
  Mux7/1 -> Goto174/1
  From326/1 -> Delay22/1
  From320/1 -> Delay21/1
  From318/1 -> Mux9/2
  From317/1 -> Mux8/2
  From315/1 -> Mux6/2
  From314/1 -> Mux7/2
  From328/1 -> Mux7/1, Mux6/1, Mux8/1, Mux9/1
  Convert3/1 -> Mux9/3, Mux8/3
  Delay21/1 -> Mux6/3
  Delay22/1 -> Mux7/3
  From321/1 -> Convert3/1
  Mux11/1 -> Goto187/1
  From519/1 -> Delay24/1
  Convert2/1 -> Mux12/3
  From342/1 -> Mux11/2
  From332/1 -> Mux11/1, Mux10/1, Mux12/1, Mux13/1
  Mux10/1 -> Goto188/1
  From341/1 -> Mux10/2
  From340/1 -> Mux13/2
  From338/1 -> Mux12/2
  Mux13/1 -> Goto190/1
  Mux12/1 -> Goto189/1
  Delay24/1 -> Mux11/3
  pipeline148/1(q) -> [ts_tvg_en]
  control/16(in_ts_tvg_en) -> pipeline148/1(d)
  pipeline3/1(q) -> [sys_rst]
  control/21(in_local_time_capture) -> edge_detect6/1(in)
  pipeline6/1(q) -> [gbe_rst]
  control/24(in_pipeline_stall) -> pipeline155/1(d)
  pipeline9/1(q) -> [gbe_stopmux]
  control/12(in_unpack_debug_reset) -> pipeline52/1(d)
  pipeline47/1(q) -> [time_diff_check_en]
  control/18(in_snap_stop_mux_sel) -> pipeline127/1(d)
  pipeline52/1(q) -> [up_dbg_rst]
  control/2(in_status_clr) -> edge_detect4/1(in)
  control/11(in_ct_tvg_en) -> pipeline59/1(d)
  control/13(in_cd_bypass) -> pipeline131/1(d)
  edge_detect1/1(out) -> pipeline14/1(d)
  control/3(in_gbe_rst) -> pipeline6/1(d)
  control/15(in_pfb_bypass) -> pipeline66/1(d)
  pipeline2/1(q) -> [force_gbe_txen]
  pipeline38/1(q) -> [gbe_cnt_rst]
  pipeline131/1(q) -> [cd_bypass]
  control/6(in_tvg_adc1) -> pipeline93/1(d)
  edge_detect6/1(out) -> pipeline164/1(d)
  pipeline43/1(q) -> [adc_snap_arm]
  control/10(in_adc_snap_trig_select) -> pipeline39/1(d)
  pipeline59/1(q) -> [ct_tvg_en]
  pipeline127/1(q) -> [snap_stop_mux_sel]
  pipeline66/1(q) -> [pfb_bypass]
  pipeline5/1(q) -> [clr_status]
  pipeline39/1(q) -> [adc_snap_trig_source]
  control/5(in_tvg_adc0) -> pipeline13/1(d)
  pipeline155/1(q) -> [pipeline_stall]
  pipeline10/1(q) -> [local_time_src]
  control/1(in_sys_rst) -> pipeline3/1(d)
  pipeline132/1(q) -> [auto_rst_enable]
  control/23(in_auto_rst_enable) -> pipeline132/1(d)
  control/22(in_time_diff_check_en) -> pipeline47/1(d)
  pipeline14/1(q) -> [cnt_rst]
  control/20(in_local_time_source) -> pipeline10/1(d)
  pipeline7/1(q) -> [gbe_txen]
  pipeline93/1(q) -> [tvg_adc1_en]
  control/14(in_gbe_stopmux) -> pipeline9/1(d)
  edge_detect2/1(out) -> pipeline38/1(d)
  control/9(in_adc_snap_arm) -> pipeline43/1(d)
  control/4(in_gbe_txen) -> pipeline7/1(d)
  pipeline128/1(q) -> [snap_reord_mux_we_sel]
  pipeline13/1(q) -> [tvg_adc0_en]
  control/19(in_snap_reord_mux_we_sel) -> pipeline128/1(d)
  control/7(in_cnt_rst) -> edge_detect1/1(in)
  control/17(in_force_gbe_txen) -> pipeline2/1(d)
  control/8(in_gbe_cnt_rst) -> edge_detect2/1(in)
  edge_detect4/1(out) -> pipeline5/1(d)
  pipeline164/1(q) -> [local_time_capture]
  control/25(in_ddc_bypass) -> pipeline1/1(d)
  control/26(in_fd_bypass) -> pipeline4/1(d)
  pipeline4/1(q) -> [fd_bypass]
  pipeline1/1(q) -> [ddc_bypass]
  Delay23/1 -> Mux10/3
  Convert4/1 -> Mux13/3
  From524/1 -> Convert4/1
  From521/1 -> Convert2/1
  we_delay15/1(q) -> snap_ctout/7(in_time_diff)
  Delay25/1 -> Logical11/1, we_delay2/1(d)
  snap_ctout/1(arm_out) -> Goto_pfb_sync30/1
  From289/1 -> snap_qout/7(arm)
  Slice24/1 -> we_delay15/1(d)
  From388/1 -> pipeline22/1(d)
  Counter17/1 -> quant_sync_cnt/1(out_reg)
  pipeline22/1(q) -> Counter17/1
  From393/1 -> pipeline21/1(d)
  pipeline21/1(q) -> Counter17/2
  pipeline49/1(q) -> Counter26/2
  From397/1 -> pipeline50/1(d)
  pipeline50/1(q) -> Counter26/1
  Counter26/1 -> cd_sync_cnt/1(out_reg)
  From399/1 -> pipeline49/1(d)
  we_delay35/1(q) -> sync_lat_tlcd_free/1(out_count)
  Counter35/1 -> Register26/1
  Register26/1 -> we_delay35/1(d)
  From416/1 -> Register26/2, Counter35/1
  From422/1 -> edge_detect13/1(in)
  edge_detect13/1(out) -> Register26/3
  From442/1 -> Register37/2, Counter46/1
  edge_detect29/1(out) -> Register37/3
  we_delay54/1(q) -> sync_lat_ct_free/1(out_count)
  From441/1 -> edge_detect29/1(in)
  Register37/1 -> we_delay54/1(d)
  Counter46/1 -> Register37/1
  Counter47/1 -> Register38/1
  Register38/1 -> we_delay55/1(d)
  From443/1 -> edge_detect30/1(in)
  we_delay55/1(q) -> sync_lat_pack_free/1(out_count)
  edge_detect30/1(out) -> Register38/3
  From445/1 -> Counter47/1, Register38/2
  edge_detect31/1(out) -> Register40/3
  From449/1 -> edge_detect31/1(in)
  From448/1 -> Register40/2
  Register40/1 -> we_delay57/1(d)
  we_delay57/1(q) -> sync_latch_tlcd/1(out_count)
  From450/1 -> Slice25/1
  Slice25/1 -> Register40/1
  Register51/1 -> we_delay68/1(d)
  we_delay68/1(q) -> sync_latch_ct/1(out_count)
  Slice37/1 -> Register51/1
  edge_detect42/1(out) -> Register51/3
  From473/1 -> Slice37/1
  From480/1 -> Register51/2
  From481/1 -> edge_detect42/1(in)
  edge_detect43/1(out) -> Register52/3
  Slice38/1 -> Register52/1
  we_delay69/1(q) -> sync_latch_pack/1(out_count)
  Register52/1 -> we_delay69/1(d)
  From482/1 -> Register52/2
  From483/1 -> edge_detect43/1(in)
  From484/1 -> Slice38/1
  fd_nb0/2(dout) -> [fd_nb_d0], Mux2/2
  From509/1 -> Convert5/1
  From510/1 -> Convert6/1
  Convert6/1 -> Mux17/3
  Delay26/1 -> Mux14/3
  Logical34/1 -> Delay26/1
  Slice43/1 -> Logical34/2
  Slice42/1 -> Logical34/1
  Counter53/1 -> Slice42/1, Slice43/1
  From511/1 -> Counter53/2
  Delay27/1 -> Mux15/3
  Mux16/1 -> Goto194/1
  Mux17/1 -> Goto195/1
  From513/1 -> Mux16/2
  From419/1 -> Mux17/2
  From493/1 -> Mux14/2
  Mux14/1 -> Goto193/1
  From512/1 -> Mux17/1, Mux16/1, Mux14/1, Mux15/1
  From502/1 -> Mux15/2
  Convert5/1 -> Mux16/3
  From503/1 -> Delay27/1, Counter53/1
  Mux15/1 -> Goto192/1
  From520/1 -> Delay23/1
  control/27(in_q_bypass) -> pipeline53/1(d)
  pipeline53/1(q) -> [q_bypass]
  edge_detect53/1(out) -> Register64/3
  Register5/1 -> edge_detect53/1(in), Logical18/1
  Counter49/1 -> Register64/1
  Logical18/1 -> Counter49/2
  Register64/1 -> Slice24/1, we_delay1/1(d)
  From301/1 -> Logical18/2
  From131/1 -> Register64/2, Counter49/1, Register5/1, Register5/3
  From246/1 -> Register5/2
  edge_detect54/1(out) -> Register65/3
  Register39/1 -> edge_detect54/1(in), Logical31/1
  Counter48/1 -> Register65/1
  Logical31/1 -> Counter48/2
  Register65/1 -> we_delay56/1(d)
  From447/1 -> Logical31/2
  From444/1 -> Register65/2, Counter48/1, Register39/1, Register39/3
  From446/1 -> Register39/2
  we_delay56/1(q) -> sync_lat_pack/1(out_count)
  edge_detect63/1(out) -> Register74/3
  Register18/1 -> edge_detect63/1(in), Logical23/1
  Counter27/1 -> Register74/1
  Logical23/1 -> Counter27/2
  Register74/1 -> we_delay25/1(d)
  From400/1 -> Logical23/2
  From402/1 -> Register74/2, Counter27/1, Register18/1, Register18/3
  From403/1 -> Register18/2
  we_delay25/1(q) -> sync_lat_tlcd/1(out_count)
  [tg_rd_sync] -> edge_detect64/1(in)
  [sync80] -> Register76/2, Register75/2
  edge_detect64/1(out) -> Register76/3, Register75/3
  Register76/1 -> we_delay77/1(d)
  spectrum_ctr7/1 -> Register76/1
  spectrum_ctr8/1 -> Register75/1
  we_delay77/1(q) -> sync_time_gen_cd_msw/1(out_msw)
  [tg_rd_time_out] -> spectrum_ctr8/1, spectrum_ctr7/1
  we_delay78/1(q) -> sync_time_gen_cd_lsw/1(out_lsw)
  Register75/1 -> we_delay78/1(d)
  [time80] -> time_gen_4/3(wr_val_in)
  time_gen_4/1(rd_sync_out) -> [tg_dds_sync]
  time_gen_4/2(rd_dvalid) -> [tg_dds_dvalid]
  time_gen_4/4(rd_misc_out) -> bus_expand13/1(bus_in)
  we_delay80/1(q) -> sync_time_pack/1(out_lsw)
  From351/1 -> Register77/2
  edge_detect65/1(out) -> Register77/3
  Register77/1 -> we_delay80/1(d)
  From350/1 -> Register77/1
  From356/1 -> edge_detect65/1(in)
  we_delay81/1(q) -> sync_time_q_lsw/1(out_lsw)
  From530/1 -> time_gen_3/4(rd_sync_in)
  From531/1 -> time_gen_3/5(rd_en)
  From527/1 -> Register78/2, Register79/2
  From_pfb_d15/1 -> time_gen_3/3(wr_val_in)
  edge_detect66/1(out) -> Register78/3, Register79/3
  From528/1 -> time_gen_3/1(wr_sync_in)
  Register79/1 -> we_delay79/1(d)
  time_gen_3/3(rd_val_out) -> spectrum_ctr9/1, spectrum_ctr12/1
  Register78/1 -> we_delay81/1(d)
  we_delay79/1(q) -> sync_time_q_msw/1(out_msw)
  From529/1 -> time_gen_3/2(wr_en)
  spectrum_ctr12/1 -> Register78/1
  spectrum_ctr9/1 -> Register79/1
  Constant13/1 -> time_gen_3/6(rd_misc_in)
  time_gen_3/1(rd_sync_out) -> edge_detect66/1(in)
  [ddc_sync] -> nb_pfb/1(sync)
  [ddc_pol0] -> nb_pfb/2(pol0)
  [ddc_pol1] -> nb_pfb/3(pol1)
  [ddc_dvalid] -> nb_pfb/4(dvalid)
  [fdfs_dv] -> Delay50/1, pipeline45/1(d)
  [fdfs_d144_1] -> Delay34/1
  [fdfs_sync] -> Delay53/1, pipeline48/1(d)
  [fdfs_dv] -> Delay52/1, pipeline41/1(d)
  [fdfs_d144_0] -> Delay2/1
  [fdfs_sync] -> Delay51/1, pipeline42/1(d)
  [q_sync] -> hmc_ct/1(in_sync)
  [q_dv] -> hmc_ct/2(in_dv)
  [q_d64_0] -> hmc_ct/3(in_d0)
  [q_d64_1] -> hmc_ct/4(in_d1)
  calc_ddc_pwr0/1(mean_pwr) -> ddc_pwr0/1(out_reg)
  [ddc_dvalid] -> Delay28/1
  Delay29/1 -> calc_ddc_pwr0/1(adc_in)
  Delay28/1 -> calc_ddc_pwr0/2(valid_in)
  [ddc_pol0] -> Delay29/1
  [ddc_pol1] -> Delay68/1
  Delay30/1 -> calc_ddc_pwr1/2(valid_in)
  Delay68/1 -> calc_ddc_pwr1/1(adc_in)
  [ddc_dvalid] -> Delay30/1
  calc_ddc_pwr1/1(mean_pwr) -> ddc_pwr1/1(out_reg)
  Constant6/1 -> cnt_rst/1(sim_1)
  Delay138/1 -> Delay134/1
  Gateway Out73/1 -> To Workspace73/1
  From359/1 -> Register7/2
  pipeline87/1(q) -> snap_acc/3(trig)
  acc_len/1(in_reg) -> pipeline70/1(d)
  Delay70/1 -> acc_cntrl1/2(sync)
  From305/1 -> pipeline46/1(d)
  Logical19/1 -> acc_cntrl1/3(rst)
  Gateway Out78/1 -> To Workspace78/1
  pipeline182/1(q) -> Gateway Out73/1, ri_to_c/2
  Constant79/1 -> acc_len/1(sim_1)
  Gateway Out69/1 -> To Workspace68/1
  pipeline86/1(q) -> Gateway Out79/1, snap_acc/2(we)
  Gateway Out58/1 -> To Workspace58/1
  Delay136/1 -> Delay129/1
  Reinterpret6/1 -> pipeline84/1(d)
  Delay73/1 -> pipeline87/1(d)
  simple_bram_vacc1/2(valid) -> spect_cnt1/2, pipeline81/1(d)
  Gateway Out59/1 -> To Workspace59/1
  pipeline67/1(q) -> Goto199/1
  From308/1 -> pipeline68/1(d)
  Delay129/1 -> Logical19/1, Gateway Out75/1, Delay70/1
  pipeline69/1(q) -> Delay137/1
  Delay111/1 -> Delay132/1
  pipeline84/1(q) -> Gateway Out78/1, snap_acc/1(in_acc)
  From309/1 -> pipeline182/1(d)
  pipeline68/1(q) -> Gateway Out72/1, ri_to_c/1
  From371/1 -> pipeline77/1(d), Gateway Out76/1, pipeline89/1(d)
  From302/1 -> acc_cntrl1/1(acc_len)
  pipeline78/1(q) -> pipeline83/1(d)
  pipeline70/1(q) -> Gateway Out68/1, Goto159/1
  From311/1 -> Logical19/2
  Delay137/1 -> Delay136/1
  pipeline46/1(q) -> Gateway Out59/1, Delay109/1
  Delay75/1 -> Delay76/1
  Gateway Out60/1 -> To Workspace60/1
  Gateway Out56/1 -> To Workspace56/1
  Slice23/1 -> Gateway Out67/1, Goto156/1
  Gateway Out77/1 -> To Workspace77/1
  pipeline60/1(q) -> pipeline54/1(d)
  From348/1 -> Delay72/1
  Delay76/1 -> Gateway Out57/1, Delay108/1
  Delay109/1 -> Delay111/1
  From307/1 -> convert/1(in)
  Delay108/1 -> acc_cntrl1/4(dvalid)
  Gateway Out57/1 -> To Workspace57/1
  bus_expand10/1(msb_out2) -> Goto200/1
  From312/1 -> pipeline69/1(d)
  pipeline54/1(q) -> simple_bram_vacc1/3(dvalid), Gateway Out80/1
  Delay132/1 -> Delay135/1
  pipeline77/1(q) -> Gateway Out66/1, spect_cnt1/1
  Gateway Out64/1 -> To Workspace65/1
  simple_bram_vacc1/1(dout) -> pipeline61/1(d), Gateway Out64/1
  bus_expand10/2(lsb_out1) -> Goto201/1
  Delay134/1 -> power1/1
  Register7/1 -> Delay69/1
  cnt_rst/1(in_reg) -> pipeline88/1(d)
  Gateway Out70/1 -> To Workspace70/1
  pipeline88/1(q) -> Slice23/1
  Gateway Out71/1 -> To Workspace71/1
  Delay74/1 -> Delay75/1
  Gateway Out66/1 -> To Workspace64/1
  Delay69/1 -> edge_detect/1
  pipeline89/1(q) -> pipeline123/1(d)
  Gateway Out72/1 -> To Workspace72/1
  From352/1 -> Delay73/1
  Gateway Out67/1 -> To Workspace66/1
  Gateway Out74/1 -> To Workspace74/1
  convert/1(out) -> Reinterpret6/1
  From304/1 -> pipeline23/1(d)
  From365/1 -> Gateway Out69/1
  From366/1 -> Gateway Out71/1
  From303/1 -> pipeline82/1(d)
  acc_cntrl1/1(new_acc) -> Goto157/1
  Gateway Out68/1 -> To Workspace67/1
  spect_cnt1/1 -> pipeline67/1(d)
  ri_to_c/1 -> Gateway Out63/1, Delay138/1
  pipeline61/1(q) -> Goto197/1
  Delay135/1 -> pipeline60/1(d)
  pipeline83/1(q) -> simple_bram_vacc1/2(din), Gateway Out77/1
  From367/1 -> Gateway Out70/1
  Gateway Out63/1 -> To Workspace63/1
  From306/1 -> Register7/3, Register7/1
  power1/1 -> Gateway Out74/1, Delay71/1
  edge_detect/1 -> Goto115/1, Gateway Out60/1
  Gateway Out79/1 -> To Workspace79/1
  Gateway Out76/1 -> To Workspace76/1
  From360/1 -> bus_expand10/1(bus_in)
  Delay72/1 -> pipeline86/1(d)
  Gateway Out75/1 -> To Workspace75/1
  pipeline81/1(q) -> Goto198/1
  pipeline82/1(q) -> simple_bram_vacc1/1(new_acc), Gateway Out58/1
  Gateway Out80/1 -> To Workspace80/1
  pipeline23/1(q) -> Gateway Out56/1, Delay74/1
  Delay71/1 -> pipeline78/1(d)
  pipeline123/1(q) -> Goto202/1
  tvg1/1(data256) -> Mux1/3
  nb_pfb/6(pfb_ch_out) -> Gateway Out14/1, Convert7/1
  Delay130/1 -> [pfb_data_out_0]
  Delay127/1 -> [pfb_sync]
  Delay128/1 -> [pfb_dv]
  Delay131/1 -> [pfb_data_out_1]
  Delay133/1 -> [pfb_of]
  Constant85/1 -> pfb_ch_inject/1(sim_1)
  pfb_ch_inject/1(in_en) -> pipeline129/1(d)
  [pfb_ch_out] -> pipeline133/1(d)
  pipeline133/1(q) -> Delay139/1
  Delay139/1 -> Delay140/1
  Mux2/1 -> demux/3(pol0_in)
  Delay140/1 -> Delay141/1
  Delay141/1 -> Gateway Out8/1, Mux2/3
  Delay142/1 -> demux/2(dv_in)
  Delay143/1 -> demux/1(sync_in)
  Delay144/1 -> demux/4(pol1_in)
  [flag_sync] -> pipeline185/1(d)
  [flag_misc] -> bus_expand11/1(bus_in)
  [flag_pktstart] -> pipeline190/1(d)
  [flag_pktxindex] -> pipeline188/1(d)
  [flag_pktfreq] -> pipeline189/1(d)
  [flag_pktxoffset] -> pipeline187/1(d)
  [flag_time] -> pipeline186/1(d)
  Delay145/1 -> snap_pack/11(trig)
  Delay146/1 -> snap_pack/10(we)
  Delay147/1 -> Gateway Out26/1, snap_pack/9(in_time)
  Delay148/1 -> Gateway Out25/1, snap_pack/8(in_sync)
  Delay149/1 -> Gateway Out24/1, snap_pack/7(in_dv)
  Delay150/1 -> Gateway Out23/1, snap_pack/6(in_pktoffset)
  Delay151/1 -> Gateway Out22/1, snap_pack/5(in_pktindex)
  Delay152/1 -> Gateway Out21/1, snap_pack/4(in_pktfreq)
  Delay153/1 -> Gateway Out20/1, snap_pack/3(in_pktstart)
  Delay154/1 -> Gateway Out19/1, snap_pack/1(in_d0)
  Constant7/1 -> pack_dv_sel/1(sim_1)
  pipeline179/1(q) -> Mux3/1
  xeng_match/1(in_val) -> pipeline184/1(d)
  pipeline156/1(q) -> match/2(data)
  pipeline158/1(q) -> data_change/1(data)
  pipeline183/1(q) -> data_change2/2(dv)
  Constant18/1 -> xeng_match/1(sim_1)
  data_change/1(trig) -> Logical20/2, Mux3/2
  pipeline168/1(q) -> data_change/2(dv)
  Reinterpret7/1 -> pipeline181/1(d)
  pipeline139/1(q) -> match/1(dv)
  Logical20/1 -> Mux3/7
  data_change2/1(trig) -> Mux3/5
  match/1(Out1) -> Logical20/1, Mux3/6
  pipeline184/1(q) -> match/3(match_value)
  Mux3/1 -> Delay149/1, Delay146/1
  pipeline177/1(q) -> data_change1/1(data)
  pipeline180/1(q) -> Delay155/1
  pack_dv_sel/1(in_sel) -> pipeline179/1(d)
  pipeline181/1(q) -> data_change2/1(data)
  pipeline178/1(q) -> data_change1/2(dv)
  data_change1/1(trig) -> Mux3/3
  Delay155/1 -> Mux3/4
  [flag_pktxindex] -> pipeline156/1(d)
  [flag_pktfreq] -> pipeline158/1(d)
  [flag_pktxindex] -> pipeline177/1(d)
  [flag_dvalid] -> pipeline178/1(d), pipeline180/1(d), pipeline183/1(d), pipeline139/1(d), pipeline168/1(d)
  [flag_pktstart] -> Reinterpret7/1
  Delay156/1 -> Delay163/1
  Delay157/1 -> Delay164/1
  Delay158/1 -> Delay165/1
  Delay159/1 -> Delay166/1
  Delay160/1 -> Delay167/1
  Delay161/1 -> Delay168/1
  Delay162/1 -> Delay169/1
  pipeline185/1(q) -> Delay156/1
  pipeline186/1(q) -> Delay157/1
  pipeline187/1(q) -> Delay158/1
  pipeline188/1(q) -> Delay159/1
  pipeline189/1(q) -> Delay160/1
  pipeline190/1(q) -> Delay161/1
  Delay163/1 -> Delay145/1, Delay148/1
  Delay164/1 -> Delay147/1
  pipeline191/1(q) -> Delay162/1
  Delay165/1 -> Delay150/1
  Delay166/1 -> Delay151/1
  Delay167/1 -> Delay152/1
  Delay168/1 -> Delay153/1
  pipeline129/1(q) -> [pfb_ch_inject]
  [pfb_ch_inject] -> Mux2/1
  bus_expand14/4(out5) -> Gateway Out114/1, Convert9/1
  Gateway Out112/1 -> To Workspace112/1
  Gateway Out115/1 -> To Workspace115/1
  Convert10/1 -> Gateway Out111/1, Concat2/3
  Gateway Out111/1 -> To Workspace111/1
  Convert9/1 -> Gateway Out110/1, Concat2/2
  Gateway Out116/1 -> To Workspace116/1
  Gateway Out109/1 -> To Workspace109/1
  Convert11/1 -> Gateway Out112/1, Concat2/4
  Gateway Out114/1 -> To Workspace114/1
  Gateway Out113/1 -> To Workspace113/1
  bus_expand14/8(lsb_out1) -> Gateway Out116/1, Convert11/1
  bus_expand14/6(out3) -> Gateway Out115/1, Convert10/1
  [fdfs_d144_0] -> bus_expand14/1(bus_in)
  Convert8/1 -> Gateway Out109/1, Concat2/1
  Concat2/1 -> Delay170/1
  bus_expand14/2(out7) -> Gateway Out113/1, Convert8/1
  Gateway Out110/1 -> To Workspace110/1
  quant0/2(dout) -> Mux4/2
  quant0/3(dvalid) -> Delay171/1
  Delay170/1 -> Mux5/3, Mux4/3
  [pfb_ch_inject] -> Mux4/1
  quant0/4(of) -> Delay172/1
  quant0/1(sync_out) -> Delay173/1
  Delay173/1 -> Gateway Out3/1, [q_sync]
  Mux4/1 -> Gateway Out5/1, [q_d64_0]
  Delay172/1 -> [q_of0]
  Delay171/1 -> Gateway Out6/1, [q_dv]
  Mux5/1 -> [q_d64_1]
  quant1/4(of) -> Delay174/1
  Delay174/1 -> [q_of1]
  quant1/2(dout) -> Mux5/2
  [pfb_ch_inject] -> Mux5/1
  Gateway Out3/1 -> To Workspace4/1
  Gateway Out5/1 -> To Workspace5/1
  Gateway Out6/1 -> To Workspace6/1
  Gateway Out8/1 -> To Workspace8/1
  Gateway Out9/1 -> To Workspace9/1
  Gateway Out10/1 -> To Workspace10/1
  Gateway Out11/1 -> To Workspace11/1
  Convert7/1 -> [pfb_ch_out]
  Gateway Out12/1 -> To Workspace12/1
  [pfb_sync] -> Gateway Out12/1
  [pfb_dv] -> Gateway Out11/1
  Gateway Out13/1 -> To Workspace13/1
  [pfb_ch_out] -> Gateway Out13/1
  Gateway Out14/1 -> To Workspace14/1
  Gateway Out15/1 -> To Workspace15/1
  Gateway Out16/1 -> To Workspace16/1
  Gateway Out17/1 -> To Workspace17/1
  Gateway Out18/1 -> To Workspace18/1
  Gateway Out19/1 -> To Workspace19/1
  Delay169/1 -> Delay154/1
  Gateway Out20/1 -> To Workspace20/1
  Gateway Out21/1 -> To Workspace21/1
  Gateway Out22/1 -> To Workspace22/1
  Gateway Out23/1 -> To Workspace23/1
  Gateway Out24/1 -> To Workspace24/1
  Gateway Out25/1 -> To Workspace25/1
  Gateway Out26/1 -> To Workspace26/1
  Delay175/1 -> snap_pack/2(in_d1)
  bus_expand11/1(msb_out8) -> bus_expand15/1(bus_in)
  bus_expand15/1(msb_out2) -> pipeline191/1(d)
  pipeline192/1(q) -> Delay176/1
  Delay176/1 -> Delay177/1
  bus_expand15/2(lsb_out1) -> pipeline192/1(d)
  Delay177/1 -> Delay175/1
  DDC/6(mix_of) -> [mix_of]
  bus_expand17/2(lsb_out1) -> pipeline195/1(d)
  bus_expand17/1(msb_out2) -> pipeline193/1(d)
  [mix_of] -> bus_expand17/1(bus_in)
  pipeline194/1(q) -> Counter13/1
  pipeline195/1(q) -> Counter13/2
  pipeline270/1(q) -> pipeline198/1(d), Counter20/1
  Counter13/1 -> pipeline197/1(d)
  Counter11/1 -> pipeline196/1(d)
  pipeline196/1(q) -> ddc_status1/3(out_mix_of0)
  pipeline197/1(q) -> ddc_status1/4(out_mix_of1)
  pipeline193/1(q) -> Counter11/2
  pipeline198/1(q) -> pipeline194/1(d), Counter11/1
  Concat17/1 -> cwg1/3(misc)
  cwg1/2(misc_out) -> bus_expand8/1(bus_in)
  [tg_dds_time_out] -> cwg1/2(time_in)
  [osc_freq] -> cwg1/1(freq)
  cwg1/1(osc_out) -> [osc_cmplx]
